simulink model "PV_SYSTEM_WITH_VARIOUS_MPPT"  (R2017a)
(part 5 of 6)

Energy-Tech (Zhejiang) ZSB-M270(156) | Solarbest Energy-Tech (Zhejiang) ZSB-P270(156) | Solarbest Energy-Tech (Zhejiang) SE-M275(156) | Solarbest Energy-Tech (Zhejiang) SE-P275(156) | Solarbest Energy-Tech (Zhejiang) ZSB-M275(156) | Solarbest Energy-Tech (Zhejiang) ZSB-P275(156) | Solarbest Energy-Tech (Zhejiang) SE-M280(156) | Solarbest Energy-Tech (Zhejiang) SE-P280(156) | Solarbest Energy-Tech (Zhejiang) ZSB-M280(156) | Solarbest Energy-Tech (Zhejiang) ZSB-P280(156) | Solarbest Energy-Tech (Zhejiang) SE-M285(156) | Solarbest Energy-Tech (Zhejiang) SE-P285(156) | Solarbest Energy-Tech (Zhejiang) ZSB-M285(156) | Solarbest Energy-Tech (Zhejiang) ZSB-P285(156) | Solarbest Energy-Tech (Zhejiang) SE-M290(156) | Solarbest Energy-Tech (Zhejiang) SE-P290(156) | Solarbest Energy-Tech (Zhejiang) ZSB-M290(156) | Solarbest Energy-Tech (Zhejiang) ZSB-P290(156) | Solarbest Energy-Tech (Zhejiang) SE-M295(156) | Solarbest Energy-Tech (Zhejiang) SE-P295(156) | Solarbest Energy-Tech (Zhejiang) ZSB-M295(156) | Solarbest Energy-Tech (Zhejiang) ZSB-P295(156) | Solarbest Energy-Tech (Zhejiang) SE-M300(156) | Solarbest Energy-Tech (Zhejiang) SE-P300(156) | Solarbest Energy-Tech (Zhejiang) ZSB-M300(156) | Solarbest Energy-Tech (Zhejiang) ZSB-P300(156) | Solarbest Energy-Tech (Zhejiang) SE-M305(156) | Solarbest Energy-Tech (Zhejiang) SE-P305(156) | Solarbest Energy-Tech (Zhejiang) ZSB-M305(156) | Solarbest Energy-Tech (Zhejiang) ZSB-P305(156) | Solarbest Energy-Tech (Zhejiang) SE-P310(156) | Solarbest Energy-Tech (Zhejiang) ZSB-P310(156) | Solarbine SB-S240TA1 | Solarbine SB-S245TA1 | Solarbine SB-S250TA1 | Solarbine S6T AC | Solarbine SB-S255TA1 | Solarbine SB-S260TA1 | Solarbine SB-S360TA1 | Solarbine SB-M365NA1 | Solarbine SB-S365TA1 | Solarbine SB-M370NA1 | Solarbine SB-S370TA1 | Solarbine SB-M375NA1 | Solarbine SB-S375TA1 | Solarbine SB-M380NA1 | Solarbine SB-S380SA1 | Solarbine SB-S380TA1 | Solarbine SB-M385NA1 | Solarbine SB-S385SA1 | Solarbine SB-S385TA1 | Solarbine SB-M390NA1 | Solarbine SB-S390SA1 | Solarbine SB-S390TA1 | Solarbine SB-M395NA1 | Solarbine SB-S395SA1 | Solarbine SB-S400SA1 | Solarbine SB-S405SA1 | Solarbine SB-S410SA1 | Solarbine SB-S415SA1 | Solarbine SB-S420SA1 | Solarfennel PS6A-230 | Solarfennel PS6A-235 | Solarfennel PS6A-240 | Solarfennel PS6A-245 | Solarfennel MS9A-250 | Solarfennel PS6A-250 | Solarfennel MS9A-255 | Solarfennel MS9A-260 | Solarfennel MS9A-265 | Solarfennel PS7A-270 | Solarfennel PS7A-275 | Solarfennel PS7A-280 | Solarfennel PS7A-285 | Solarfennel PS7A-290 | Solarfun Power SF220-30-P230 | Solarfun Power SF220-30-P235 | Solarfun Power SF220-30-P240 | Solargate Technology SG-2150 | Solargate Technology SG-2200 | Solargate Technology SG-2250 | Solargate Technology SG-2300 | Solargate Technology SG-2350 | Solaria Solaria 210 | Solaria Solaria 210 Frameless | Solaria Solaria 220 | Solaria Solaria 220 Frameless | Solaria Solaria 225 | Solaria Solaria 225 Frameless | Solaria Solaria 230 | Solaria Solaria 230 Frameless | Solaria Solaria 240 | Solaria Solaria 245 | Solaria Solaria 250 | Solaria Solaria 255 | Solaria Solaria 260 | Solaria Solaria 265 | Solaria Solaria 270 | Solaria Solaria 275 | Solaria Solaria 280 | Solarland USA SLP115S-17H | Solarland USA SLP120S-17H | Solarland USA SLP125S-17H | Solarland USA SLP160S-24H | Solarland USA SLP165S-24H | Solarland USA SLP170S-24H | Solarland USA SLP175S-24H | Solarland USA SLP175S-24J | Solarland USA SLP180S-24H | Solarland USA SLP180S-24J | Solarland USA SLP185S-24H | Solarland USA SLP185S-24J | Solarland USA SLP185S-72 | Solarland USA SLP190S-24H | Solarland USA SLP190S-72 | Solarland USA SLP195S-24H | Solarland USA SLP200-18H | Solarland USA SLP200S-24H | Solarland USA SLP205-18H | Solarland USA SLP210-18H | Solarland USA SLP215-18H | Solarland USA SLP215-60 | Solarland USA SLP220-18H | Solarland USA SLP220-60 | Solarland USA SLP225-60 | Solarland USA SLP230-18H | Solarland USA SLP230-60 | Solarland USA SLP230S-96 | Solarland USA SLP235-18H | Solarland USA SLP235-60 | Solarland USA SLP240-18H | Solarland USA SLP240S-96 | Solarland USA SLP245S-96 | Solarland USA SLP250S-96 | SolarPark Korea SPP 220 | SolarPark Korea SPP 225 | SolarPark Korea SPP 230 | SolarPark Korea SPP235 | SolarPark Korea SPP240 | SolarPark Korea SPP245 | SolarPark Korea SPP245 mono | SolarPark Korea SPP 250 | SolarPark Korea SPP250 mono | SolarPark Korea SPP255 mono | SolarPark Korea SPP260 mono | Solarpeace P6Y-230 | Solarpeace P6Y-235 | Solarpeace P6Y-240 | Solarpeace P6Y-245 | Solarpeace M9X-250 | Solarpeace P6Y-250 | Solarpeace M9X-255 | Solarpeace M9X-260 | Solarpeace M9X-265 | Solarpeace P7Y-270 | Solarpeace P7Y-275 | Solarpeace P7Y-280 | Solarpeace P7Y-285 | Solarpeace P7Y-290 | Solartec USA SDM-170-(165)-72M | Solartec USA SDM-170-(170)-72M | Solartec USA SDM-170-(175)-72M | Solartec USA SDM-170-(180)-72M | Solartec USA SDM-170-(185)-72M | Solartec S72MC-195 | Solartec S60MC-250 | Solartec S72PC-280 | Solartec S72MC6-300 | Solartech Energy ASC-6P-36-130 | Solartech Energy ASC-6P-36-135 | Solartech Energy ASC-6P-36-140 | Solartech Energy ASC-6P-36-145 | Solartech Energy ASC-6P-36-150 | Solartech Energy ASC-6P-48-175 | Solartech Energy ASC-6P-48-180 | Solartech Energy ASC-6P-48-185 | Solartech Energy ASC-6P-48-190 | Solartech Energy ASC-6P-48-195 | Solartech Energy ASC-6P-48-200 | Solartech Energy ASC-6P-54-200 | Solartech Energy ASC-6P-54-205 | Solartech Energy ASC-6P-54-210 | Solartech Energy SEC-210W-M6-G | Solartech Energy ASC-6P-54-215 | Solartech Energy SEC-215W-M6-G | Solartech Energy ASC-6P-54-220 | Solartech Energy ASC-6P-60-220 | Solartech Energy SEC-220W-M6-G | Solartech Energy SEC-6P-60-220 | Solartech Energy ASC-6P-54-225 | Solartech Energy ASC-6P-60-225 | Solartech Energy SEC-225W-M6-G | Solartech Energy SEC-6P-60-225 | Solartech Energy ASC-6P-54-230 | Solartech Energy ASC-6P-60-230 | Solartech Energy SEC-230W-M6-G | Solartech Energy SEC-6P-60-230 | Solartech Energy ASC-6P-60-235 | Solartech Energy SEC-6P-60-235 | Solartech Energy ASC-6P-60-240 | Solartech Energy SEC-6P-60-240 | Solartech Energy ASC-6P-60-245 | Solartech Energy SEC-6P-60-245 | Solartech Energy ASC-6P-60-250 | Solartech Energy ASC-6P-60-255 | Solartech Energy ASC-6P-72-265 | Solartech Energy ASC-6P-72-270 | Solartech Energy ASC-6P-72-275 | Solartech Energy ASC-6P-72-280 | Solartech Energy ASC-6P-72-285 | Solartech Energy ASC-6P-72-290 | Solartech Energy ASC-6P-72-295 | Solartech Energy ASC-6P-72-300 | Solartech Energy ASC-6P-72-305 | Solartech Power SPM190P | Solartech Power SPM195P | Solartech Power SPM200P | Solartech Power SPM205P | Solartech Power SPM210P | Solartech Power SPM220P | Solartech Power SPM225P | Solartech Power SPM230P | Solartech Power SPM235P | Solartech Power SPM240P | Solartech Renewables STR205 | Solartech Renewables STR210 | Solartech Renewables STR215 | Solartech Renewables STR220 | Solartech Renewables STR225 | Solartech Renewables STR230 | Solartechnics North America MP165Wp | Solartechnics North America Mp170Wp | Solartechnics North America MP175Wp | Solartechnics North America MP180Wp | SolarWorld SW165 mono | SolarWorld SW175 mono | SolarWorld SW220 mono | SolarWorld SW220 mono black | SolarWorld SW220 Poly | SolarWorld SW225 mono | SolarWorld SW225 mono black | SolarWorld SW225 Poly | SolarWorld SW230 mono | SolarWorld SW230 mono black | SolarWorld SW230 Poly | SolarWorld SW235 mono | SolarWorld SW235 mono black | SolarWorld SW235 Poly | SolarWorld SW240 mono | SolarWorld SW240 mono black | SolarWorld SW240 Poly | SolarWorld SW245 mono | SolarWorld SW245 Mono Black | SolarWorld SW245 Poly | SolarWorld SW250 Mono | SolarWorld SW250 Mono Black | SolarWorld SW250 Poly | SolarWorld Protect SW 255 Mono | SolarWorld Protect SW 255 Mono Black | SolarWorld SW255 Mono | SolarWorld SW255 Mono Black | SolarWorld SW255 Poly | SolarWorld Protect SW 260 Mono | SolarWorld Protect SW 260 Mono Black | SolarWorld SW260 Mono | SolarWorld SW260 Mono Black | SolarWorld Protect SW 265 Mono | SolarWorld Protect SW 265 Mono Black | SolarWorld SW265 Mono | SolarWorld SW265 Mono Black | SolarWorld Protect SW 270 Mono | SolarWorld Protect SW 270 Mono Black | SolarWorld SW270 Mono | SolarWorld SW270 Mono Black | SolarWorld Protect SW 275 Mono | SolarWorld SW275 Mono | Solarzentrum Allgau Wiosun A-170P | Solarzentrum Allgau Wiosun PVT 170 | Solarzentrum Allgau Wiosun A-175P | Solarzentrum Allgau Wiosun PVT 175 | Solarzentrum Allgau Wiosun A-180P | Solarzentrum Allgau Wiosun PVT 180 | Solarzentrum Allgau Wiosun A-185P | Solarzentrum Allgau Wiosun PVT 185 | Solarzentrum Allgau Wiosun A-190P | Solarzentrum Allgau Wiosun PVT 190 | SOLON SOLON Blue 220-01 215 | SOLON SOLON Blue 220 | SOLON SOLON Blue 220-01 220 | SOLON SOLON Black 225 | SOLON SOLON Black 230-01 225 | SOLON SOLON Black 230-15 225 | SOLON SOLON Blue 220-01 225 | SOLON SOLON Blue 225 | SOLON SOLON Corvus 225 | SOLON SOLON Black 230 | SOLON SOLON Black 230-01 230 | SOLON SOLON Black 230-15 230 | SOLON SOLON Blue 220-01 230 | SOLON SOLON Blue 230 | SOLON SOLON Corvus 230 | SOLON SOLON Black 230-01 235 | SOLON SOLON Black 230-15 235 | SOLON SOLON Black 235 | SOLON SOLON Blue 220-01 235 | SOLON SOLON Blue 235 | SOLON SOLON Corvus 235 | SOLON SOLON Black 230-01 240 | SOLON SOLON Black 230-15 240 | SOLON SOLON Black 240 | SOLON SOLON Blue 220-01 240 | SOLON SOLON Blue 240 | SOLON SOLON Corvus 240 | SOLON SOLON Black 245 | SOLON SOLON Blue 270-09 250 | SOLON SOLON Blue 270-09 255 | SOLON SOLON Blue 270-09 260 | SOLON SOLON Black 280-09 265 | SOLON SOLON Blue 270-09 265 | SOLON SOLON Blue XT 265 | SOLON SOLON Black 280-09 270 | SOLON SOLON Blue 270-09 270 | SOLON SOLON Blue XT 270 | SOLON SOLON Black 280-09 275 | SOLON SOLON Black XT 275 | SOLON SOLON Blue 270-09 275 | SOLON SOLON Blue XT 275 | SOLON SOLON Black 280-09 280 | SOLON SOLON Black XT 280 | SOLON SOLON Blue 270-09 280 | SOLON SOLON Blue XT 280 | SOLON SOLquick Black XT 280 | SOLON SOLquick Blue XT 280 | SOLON SOLquick Blue XT-H 280 | SOLON SOLON Black 280-09 285 | SOLON SOLON Black XT 285 | SOLON SOLON Blue 270-09 285 | SOLON SOLON Blue XT 285 | SOLON SOLquick Black XT 285 | SOLON SOLquick Blue XT 285 | SOLON SOLON Black 280-09 290 | SOLON SOLON Black XT 290 | SOLON SOLON Blue 270-09 290 | SOLON SOLquick Black XT 290 | SOLON SOLON Black 280-09 295 | SOLON SOLON Black XT 295 | SOLON SOLquick Black XT 295 | SOLON SOLON Black 280-09 300 | Solon SOLquick Black XT 300 | Solvation Manufacturing P6Y-230 | Solvation Manufacturing P6Y-235 | Solvation Manufacturing P6Y-240 | Solvation Manufacturing SM240-5M | Solvation Manufacturing SM240M-B | Solvation Manufacturing P6Y-245 | Solvation Manufacturing SM245-5M | Solvation Manufacturing SM245M-B | Solvation Manufacturing SM245M-Bv | Solvation Manufacturing SM245S-B | Solvation Manufacturing M9X-250 | Solvation Manufacturing P6Y-250 | Solvation Manufacturing SM250-5M | Solvation Manufacturing SM250M-B | Solvation Manufacturing SM250M-Bv | Solvation Manufacturing SM250S-B | Solvation Manufacturing M9X-255 | Solvation Manufacturing SM255-5M | Solvation Manufacturing SM255M-B | Solvation Manufacturing SM255M-Bv | Solvation Manufacturing SM255S-B | Solvation Manufacturing M9X-260 | Solvation Manufacturing SM260-5M | Solvation Manufacturing SM260M-Bv | Solvation Manufacturing M9X-265 | Solvation Manufacturing SM265M-Bv | Solvation Manufacturing P7Y-270 | Solvation Manufacturing SM270M-A | Solvation Manufacturing P7Y-275 | Solvation Manufacturing SM275M-A | Solvation Manufacturing P7Y-280 | Solvation Manufacturing SM280M-A | Solvation Manufacturing P7Y-285 | Solvation Manufacturing SM285M-A | Solvation Manufacturing SM285M-Av | Solvation Manufacturing P7Y-290 | Solvation Manufacturing SM290M-A | Solvation Manufacturing SM290M-Av | Solvation Manufacturing SM295M-A | Solvation Manufacturing SM295M-Av | Solvation Manufacturing SM300M-A | Solvation Manufacturing SM300M-Av | Solvation Manufacturing SM305M-A | Solvation Manufacturing SM305M-Av | Solvation Manufacturing SM310M-Av | Solvation Manufacturing SM315M-Av | Sonali Energees USA SS 1200 P | Sonali Energees USA SS 1250 P | Sonali Energees USA SS 1300 P | Sonali Energees USA SS 1400 P | Sonali Energees USA SS1750-170W | Sonali Energees USA SS 1750 P | Sonali Energees USA SS1750-175W | Sonali Energees USA SS 1800 P | Sonali Energees USA SS1750-180W | Sonali Energees USA SS 1900 P | Sonali Energees USA SS 2000 P | Sonali Energees USA SS 2100 P | Sonali Energees USA SS2100-210W | Sonali Energees USA SS2100-215W | Sonali Energees USA SS 2200 P | Sonali Energees USA SS2100-220W | Sonali Energees USA SS 2300 P | Sonali Energees USA SS2300-230W | Sonali Energees USA SS2300-235W | Sonali Energees USA SS 2400 P | Sonali Energees USA SS2300-240W | Sonali Energees USA SS2500-250W | Sonali Energees USA SS2800-275W | Sonali Energees USA SS2800-280W | Sonali Energees USA SS2800-285W | Sonali Energees SS 270 | Sonali Energees SS 280 | Sonali Energees SS 290 | Sonnetek SNK-165PSD | Sonnetek SNK-170PSD | Sonnetek SNK-175PSD | Sonnetek SNK-180PSD | Sonnetek SNK-250PSP | Sonnetek SNK-260PSP | Sonnetek SNK-270PSP | Sopray Energy SR-150 | Sopray Energy SR-160 | Sopray Energy SR-165 | Sopray Energy SR-170 | Sopray Energy SR-175 | Sopray Energy SR-180 | Sopray Energy SR156P-200 | Sopray Energy SR156P-210 | Sopray Energy SR156P-220 | Sopray Energy SR156P-230 | Sova Power SOLARSOVA 200P | Sova Power SOLARSOVA 205P | Sova Power SOLARSOVA 210P | Sova Power SOLARSOVA 215P | Sova Power SOLARSOVA 220P | Sova Power SOLARSOVA 235P | Sova Power SOLARSOVA 240P | Sova Power SOLARSOVA 245P | Sova Power SOLARSOVA 250P | Sova Power SOLARSOVA 255P | Sova Power SOLARSOVA 260P | Sovello SV-T-190-yyy | Sovello SV-X-190-yyy | Sovello SV-T-195-yyy | Sovello SV-X-195-yyy | Sovello SV-T-200-yyy | Sovello SV-X-200-yyy | Sovello SV-X-205-yyy | Sovello SV-X-210-yyy | SRS Energy SPT16 | Star Harvest Solar SHS260-5M | Stion SN-110 | Stion STN-110 | Stion SN-115 | Stion STN-115 | Stion SN-120 | Stion STN-120 | Stion SN-125 | Stion STN-125 | Stion STX-125 | Stion SN-130 | Stion STN-130 | Stion STX-130 | Stion SN-135 | Stion STN-135 | Stion STX-135 | Stion SN-140 | Stion STN-140 | Stion STX-140 | Stion SN-145 | Stion STN-145 | Stion STX-145 | Stion SN-150 | Stion STN-150 | STX Solar STX-240MT2 | STX Solar STX-245MT2 | STX Solar STX-250MT2 | STX Solar STX-255MT2 | STX Solar STX-260MT2 | STX Solar STX-290MT2 | STX Solar STX-295MT2 | STX Solar STX-300MT2 | STX Solar STX-305MT2 | Sun Earth Solar Power TDB125x125-36-P 80W | Sun Earth Solar Power TDB125x125-36-P 85W | Sun Earth Solar Power TPB125x125-36-P 85W | Sun Earth Solar Power TDB125x125-36-P 90W | Sun Earth Solar Power TPB125x125-36-P 90W | Sun Earth Solar Power TDB125x125-36-P 95W | Sun Earth Solar Power TPB125x125-36-P 95W | Sun Earth Solar Power TDB156x156-36-P 125W | Sun Earth Solar Power TPB156x156-36-P 125W | Sun Earth Solar Power TDB156x156-36-P 130W | Sun Earth Solar Power TPB156x156-36-P 130W | Sun Earth Solar Power TDB156x156-36-P 135W | Sun Earth Solar Power TPB156x156-36-P 135W | Sun Earth Solar Power TDB156x156-36-P 140W | Sun Earth Solar Power TPB156x156-36-P 140W | Sun Earth Solar Power TDB156x156-36-P 145W | Sun Earth Solar Power TPB156x156-36-P 145W | Sun Earth Solar Power TDB125x125-72-P 150W | Sun Earth Solar Power TPB125x125-72-P 150W | Sun Earth Solar Power TDB125x125-72-P 155W | Sun Earth Solar Power TPB125x125-72-P 155W | Sun Earth Solar Power TDB125x125-72-P 160W | Sun Earth Solar Power TPB125x125-72-P 160W | Sun Earth Solar Power TDB125x125-72-P 165W | Sun Earth Solar Power TPB125x125-72-P 165W | Sun Earth Solar Power TDB125x125-72-P 170W | Sun Earth Solar Power TPB125x125-72-P 170W | Sun Earth Solar Power TDB125x125-72-P 175W | Sun Earth Solar Power TPB125x125-72-P 175W | Sun Earth Solar Power TDB125x125-72-P 180W | Sun Earth Solar Power TPB125x125-72-P 180W | Sun Earth Solar Power TPB156x156-54-P 180W | Sun Earth Solar Power TDB125x125-72-P 185W | Sun Earth Solar Power TPB125x125-72-P 185W | Sun Earth Solar Power TPB156x156-54-P 185W | Sun Earth Solar Power TDB125x125-72-P 190W | Sun Earth Solar Power TPB125x125-72-P 190W | Sun Earth Solar Power TPB156x156-54-P 190W | Sun Earth Solar Power TPB156x156-54-P 195W | Sun Earth Solar Power TPB125x125-96-P 200W | Sun Earth Solar Power TPB156x156-54-P 200W | Sun Earth Solar Power TPB156x156-60-P 200W | Sun Earth Solar Power TPB156x156-54-P 205W | Sun Earth Solar Power TPB156x156-60-P 205W | Sun Earth Solar Power TPB125x125-96-P 210W | Sun Earth Solar Power TPB156x156-54-P 210W | Sun Earth Solar Power TPB156x156-60-P 210W | Sun Earth Solar Power TDB156x156-60-P 215W | Sun Earth Solar Power TPB156x156-54-P 215W | Sun Earth Solar Power TPB156x156-60-P 215W | Sun Earth Solar Power TDB156x156-60-P 220W | Sun Earth Solar Power TPB125x125-96-P 220W | Sun Earth Solar Power TPB156x156-54-P 220W | Sun Earth Solar Power TPB156x156-60-P 220W | Sun Earth Solar Power TDB156x156-60-P 225W | Sun Earth Solar Power TPB156x156-60-P 225W | Sun Earth Solar Power TDB156x156-60-P 230W | Sun Earth Solar Power TPB125x125-96-P 230W | Sun Earth Solar Power TPB156x156-60-P 230W | Sun Earth Solar Power TPB156x156-72-P 230W | Sun Earth Solar Power TDB156x156-60-P 235W | Sun Earth Solar Power TPB156x156-60-P 235W | Sun Earth Solar Power TDB156x156-60-P 240W | Sun Earth Solar Power TPB125x125-96-P 240W | Sun Earth Solar Power TPB156x156-60-P 240W | Sun Earth Solar Power TPB156x156-72-P 240W | Sun Earth Solar Power TDB156x156-60-P 245W | Sun Earth Solar Power TPB156x156-60-P 245W | Sun Earth Solar Power TPB156x156-72-P 250W | Sun Earth Solar Power TPB156x156-72-P 255W | Sun Earth Solar Power TPB156x156-72-P 260W | Sun Earth Solar Power TPB156x156-72-P 270W | Sun Earth Solar Power TDB156x156-72-P 280W | Sun Earth Solar Power TPB156x156-72-P 280W | Sun Earth Solar Power TDB156x156-72-P 285W | Sun Earth Solar Power TPB156x156-72-P 285W | Sun Earth Solar Power TDB156x156-72-P 290W | Sun Earth Solar Power TPB156x156-72-P 290W | Sun Earth Solar Power TDB156x156-72-P 295W | Sun Earth Solar Power TPB156x156-72-P 295W | Sun Energy Engineering SE14-50 | Sun Energy Engineering SE14-52 | Sun World Solar Energy Technology (Luoyang) SWM230P156 | Sun World Solar Energy Technology (Luoyang) SWM235M156 | Sun World Solar Energy Technology (Luoyang) SWM235P156 | Sun World Solar Energy Technology (Luoyang) SWM240M156 | Sun World Solar Energy Technology (Luoyang) SWM240P156 | Sun World Solar Energy Technology (Luoyang) SWM245M156 | Sun World Solar Energy Technology (Luoyang) SWM245P156 | Sun World Solar Energy Technology (Luoyang) SWM250M156 | Sun World Solar Energy Technology (Luoyang) SWM250P156 | Sun World Solar Energy Technology (Luoyang) SWM255M156 | Sun World Solar Energy Technology (Luoyang) SWM280P156 | Sun World Solar Energy Technology (Luoyang) SWM285M156 | Sun World Solar Energy Technology (Luoyang) SWM285P156 | Sun World Solar Energy Technology (Luoyang) SWM290M156 | Sun World Solar Energy Technology (Luoyang) SWM290P156 | Sun World Solar Energy Technology (Luoyang) SWM295M156 | Sun World Solar Energy Technology (Luoyang) SWM295P156 | Sun World Solar Energy Technology (Luoyang) SWM300M156 | Sun World Solar Energy Technology (Luoyang) SWM300P156 | Sunarray SUNARRAY-M6B2409-130 | Sunarray SUNARRAY-M6B2409-135 | Sunarray SUNARRAY-S6B2409-135 | Sunarray SUNARRAY-M6B2409-140 | Sunarray SUNARRAY-S6B2409-140 | Sunarray SUNARRAY-S6B2409-145 | Sunarray SUNARRAY-M6B2608-175 | Sunarray SUNARRAY-M6B2608-180 | Sunarray SUNARRAY-S6B2608-180 | Sunarray SUNARRAY-M6B2608-185 | Sunarray SUNARRAY-S6B2608-185 | Sunarray SUNARRAY-M6B2609-190 | Sunarray SUNARRAY-S6B2608-190 | Sunarray SUNARRAY-M6B2609-195 | Sunarray SUNARRAY-S6B2609-195 | Sunarray SUNARRAY-M6B2609-200 | Sunarray SUNARRAY-S6B2609-200 | Sunarray SUNARRAY-M6B2609-205 | Sunarray SUNARRAY-S6B2609-205 | Sunarray SUNARRAY-M6B2609-210 | Sunarray SUNARRAY-S6B2609-210 | Sunarray SUNARRAY-M6B2609-215 | Sunarray SUNARRAY-S6B2609-215 | Sunarray SUNARRAY-M6B2609-220 | Sunarray SUNARRAY-S6B2609-220 | Sunarray SUNARRAY-M6B2609-225 | Sunarray SUNARRAY-S6B2609-225 | Sunarray SUNARRAY-M6B2609-230 | Sunarray SUNARRAY-S6B2609-230 | Sunarray SUNARRAY-M6B2610-235 | Sunarray SUNARRAY-S6B2609-235 | Sunarray SUNARRAY-M6B2610-240 | Sunarray SUNARRAY-S6B2609-240 | Sunarray SUNARRAY-M6B3612-270T | Sunarray SUNARRAY-M6B2612-275 | Sunarray SUNARRAY-M6B3612-275T | Sunarray SUNARRAY-M6B2612-280 | Sunarray SUNARRAY-M6B3612-280T | Sunarray SUNARRAY-M6B2612-285 | Sunarray SUNARRAY-M6B3612-285T | Sunarray SUNARRAY-S6B3612-285T | Sunarray SUNARRAY-M6B2612-290 | Sunarray SUNARRAY-M6B3612-290T | Sunarray SUNARRAY-S6B3612-290T | Sunarray SUNARRAY-M6B2612-295 | Sunarray SUNARRAY-S6B3612-295T | Sunarray SUNARRAY-S6B3612-300T | Sunarray SUNARRAY-S6B3612-305T | SUNGEN International SG-HN90-GG | SUNGEN International SG-HN95-GG | SUNGEN International SG-HN100-GG | SUNGEN International SG-HN105-GG | SUNGEN International SG-HN110-GG | SUNGEN International SGM-160D | SUNGEN International SGM-165D | SUNGEN International SGM-170D | SUNGEN International SGM-175D | SUNGEN International SGM-180D | SUNGEN International SGM-185D | SUNGEN International SGM-190D | SUNGEN International SGM-195D | SUNGEN International SGM-200D | SUNGEN International SGM-200P | SUNGEN International SGM-205D | SUNGEN International SGM-205P | SUNGEN International SGM-210D | SUNGEN International SGM-210P | SUNGEN International SGM-215D | SUNGEN International SGM-215P | SUNGEN International SGM-220D | SUNGEN International SGM-220P | SUNGEN International SGM-225D | SUNGEN International SGM-225P | SUNGEN International SGM-230D | SUNGEN International SGM-230P | SUNGEN International SGM-235D | SUNGEN International SGM-235P | SUNGEN International SGM-240D | SUNGEN International SGM-240P | SUNGEN International SGM-245D | SUNGEN International SGM-245P | SUNGEN International SGM-250D | SUNGEN International SGM-250P | SUNGEN International SGM-255P | SUNGEN International SGM-260D | SUNGEN International SGM-260P | SUNGEN International SGM-265P | SUNGEN International SGM-270P | SUNGEN International SGM-275P | SUNGEN International SGM-280P | SUNGEN International SGM-285P | Suniva MVS220-60-5-501 | Suniva MVS225-60-5-501 | Suniva ART230-60-3-100 | Suniva MVP230-60-5-401 | Suniva MVS230-60-5-501 | Suniva ART235-60-3-100 | Suniva ART235-60-3-101 | Suniva ART235-60-3-1B0 | Suniva MVP235-60-5-401 | Suniva MVS235-60-5-501 | Suniva MVT235-60-5-100 | Suniva MVX235-60-5-701 | Suniva OPT235-60-4-100 | Suniva OPT235-60-4-1B0 | Suniva ART240-60-3-100 | Suniva ART240-60-3-101 | Suniva ART240-60-3-1B0 | Suniva MVP240-60-5-401 | Suniva MVS240-60-5-501 | Suniva MVT240-60-5-100 | Suniva MVX240-60-5-701 | Suniva MVX240-60-5-7B1 | Suniva MVX240-60-5-801 | Suniva MVX240-60-5-8B1 | Suniva OPT240-60-4-100 | Suniva OPT240-60-4-1B0 | Suniva ART245-60-3-100 | Suniva ART245-60-3-101 | Suniva ART245-60-3-1B0 | Suniva MVT245-60-5-100 | Suniva MVX245-60-5-701 | Suniva MVX245-60-5-7B1 | Suniva MVX245-60-5-801 | Suniva MVX245-60-5-8B1 | Suniva OPT245-60-4-100 | Suniva OPT245-60-4-1B0 | Suniva ART250-60-3-100 | Suniva ART250-60-3-101 | Suniva ART250-60-3-1B0 | Suniva MVT250-60-5-100 | Suniva MVX250-60-5-701 | Suniva MVX250-60-5-7B1 | Suniva MVX250-60-5-801 | Suniva MVX250-60-5-8B1 | Suniva OPT250-60-4-100 | Suniva OPT250-60-4-1B0 | Suniva OPT250-60-4-700 | Suniva OPT250-60-4-7B0 | Suniva OPT250-60-4-800 | Suniva OPT250-60-4-8B0 | Suniva ART255-60-3-100 | Suniva ART255-60-3-1B0 | Suniva MVX255-60-5-701 | Suniva MVX255-60-5-7B1 | Suniva MVX255-60-5-801 | Suniva MVX255-60-5-8B1 | Suniva OPT255-60-4-100 | Suniva OPT255-60-4-1B0 | Suniva OPT255-60-4-700 | Suniva OPT255-60-4-7B0 | Suniva OPT255-60-4-800 | Suniva OPT255-60-4-8B0 | Suniva MVX260-60-5-7B1 | Suniva MVX260-60-5-801 | Suniva MVX260-60-5-8B1 | Suniva OPT260-60-4-100 | Suniva OPT260-60-4-1B0 | Suniva OPT260-60-4-700 | Suniva OPT260-60-4-7B0 | Suniva OPT265-60-4-100 | Suniva OPT265-60-4-1B0 | Suniva OPT270-60-4-100 | Suniva MVP280-72-5-401 | Suniva MVT280-72-5-100 | Suniva MVP285-72-5-401 | Suniva MVT285-72-5-100 | Suniva MVX285-72-5-701 | Suniva MVX285-72-5-801 | Suniva MVT290-72-5-100 | Suniva MVX290-72-5-701 | Suniva MVX290-72-5-801 | Suniva OPT290-72-4-100 | Suniva MVT295-72-5-100 | Suniva MVX295-72-5-701 | Suniva MVX295-72-5-801 | Suniva OPT295-72-4-100 | Suniva MVT300-72-5-100 | Suniva MVX300-72-5-701 | Suniva MVX300-72-5-801 | Suniva OPT300-72-4-100 | Suniva MVX305-72-5-701 | Suniva MVX305-72-5-801 | Suniva OPT305-72-4-100 | Suniva OPT305-72-4-800 | Suniva MVX310-72-5-801 | Suniva OPT310-72-4-100 | Suniva OPT310-72-4-800 | Suniva OPT315-72-4-100 | Suniva OPT315-72-4-800 | Suniva OPT320-72-4-800 | Sunlan Solar SLM225P | Sunlan Solar SLM230P | Sunlan Solar SLM235P | Sunlan Solar SLM240P | Sunlan Solar SLM245P | Sunlan Solar SLM270P | Sunlan Solar SLM275P | Sunlan Solar SLM280P | Sunny International Power SPM-180PB203 | Sunny International Power SPM-180SB105 | Sunny International Power SPM-190PB203 | Sunny International Power SPM-190SB105 | Sunny International Power SPM-200PB203 | Sunny International Power SPM-200PB204 | Sunny International Power SPM-200SB105 | Sunny International Power SPM-210PB203 | Sunny International Power SPM-210PB204 | Sunny International Power SPM-220PB203 | Sunny International Power SPM-220PB204 | Sunny International Power SPM-230PB204 | Sunny International Power SPM-230PB206 | Sunny International Power SPM-240PB204 | Sunny International Power SPM-240PB205 | Sunny International Power SPM-240PB206 | Sunny International Power SPM-250PB205 | Sunny International Power SPM-250PB206 | Sunny International Power SPM-260PB205 | Sunny International Power SPM-260PB206 | Sunny International Power SPM-270PB205 | Sunny International Power SPM-270PB206 | Sunny International Power SPM-280PB205 | Sunny International Power SPM-290PB205 | Sunny Optronics 7NACF00-06A225 | Sunny Optronics 7NACF00-06A230 | Sunny Optronics 7NACF00-06A235 | Sunny Optronics 7NACF00-06A240 | Sunny Optronics 7NACF00-06A245 | Sunperfect Solar CRM60S125M-24 | Sunperfect Solar CRM60S125S | Sunperfect Solar CRM85S125M-36 | Sunperfect Solar CRM85S125S | Sunperfect Solar CRM115S125M-48 | Sunperfect Solar CRM115S125S | Sunperfect Solar CRM145S125M-60 | Sunperfect Solar CRM145S125S | Sunperfect Solar CRM175S125M-72 | Sunperfect Solar CRM175S125S | Sunperfect Solar CRM180S125M-72 | Sunperfect Solar CRM185S125M-72 | Sunperfect Solar CRM185S156P-54 | Sunperfect Solar CRM190S125M-72 | Sunperfect Solar CRM190S156P-54 | Sunperfect Solar CRM195S125M-72 | Sunperfect Solar CRM195S125M-80 | Sunperfect Solar CRM195S125S | Sunperfect Solar CRM195S156P-54 | Sunperfect Solar CRM200S156P-54 | Sunperfect Solar CRM200S156P-60 | Sunperfect Solar CRM205S125M-80 | Sunperfect Solar CRM205S156P-54 | Sunperfect Solar CRM205S156P-60 | Sunperfect Solar CRM210S125M-80 | Sunperfect Solar CRM210S156P-54 | Sunperfect Solar CRM210S156P-60 | Sunperfect Solar CRM215S125M-80 | Sunperfect Solar CRM215S156P-54 | Sunperfect Solar CRM215S156P-60 | Sunperfect Solar CRM220S156P-54 | Sunperfect Solar CRM220S156P-60 | Sunperfect Solar CRM225S156P-54 | Sunperfect Solar CRM225S156P-60 | Sunperfect Solar CRM230S156P-54 | Sunperfect Solar CRM230S156P-60 | Sunperfect Solar CRM235S125M-96 | Sunperfect Solar CRM235S125S | Sunperfect Solar CRM235S156P-60 | Sunperfect Solar CRM240S125M-96 | Sunperfect Solar CRM240S156P-60 | Sunperfect Solar CRM240S156P-72 | Sunperfect Solar CRM245S125M-96 | Sunperfect Solar CRM245S156P-60 | Sunperfect Solar CRM245S156P-72 | Sunperfect Solar CRM250S125M-96 | Sunperfect Solar CRM250S156P-60 | Sunperfect Solar CRM250S156P-72 | Sunperfect Solar CRM255S125M-96 | Sunperfect Solar CRM255S156P-60 | Sunperfect Solar CRM255S156P-72 | Sunperfect Solar CRM260S125M-96 | Sunperfect Solar CRM260S156P-60 | Sunperfect Solar CRM260S156P-72 | Sunperfect Solar CRM265S125M-96 | Sunperfect Solar CRM265S156P-72 | Sunperfect Solar CRM270S156P-72 | Sunperfect Solar CRM275S156P-72 | Sunperfect Solar CRM280S156P-72 | Sunperfect Solar CRM285S156P-72 | Sunperfect Solar CRM290S156P-72 | Sunperfect Solar CRM295S156P-72 | Sunperfect Solar CRM300S156P-72 | SunPower PL-PLT-63L-BLK-U | SunPower SPR-76R-BLK-U | SunPower SPR-76RE-BLK-U | SunPower SPR-200-BLK-U | SunPower SPR-200-WHT-U | SunPower SPR-205-BLK-U | SunPower SPR-208-WHT-U | SunPower SPR-210-BLK-U | SunPower SPR-210-WHT-U | SunPower PL-SUNP-SPR-215 | SunPower SPR-215-WHT-U | SunPower SPR-217-WHT-U | SunPower SER-220P | SunPower SPR-220-BLK-U | SunPower SPR-220-WHT-U | SunPower SPR-225-BLK-U | SunPower SPR-225E-BLK-D | SunPower SPR-225E-BLK-U-ACPV | SunPower SPR-225E-WHT-D | SunPower SPR-225NE-BLK-D | SunPower SER-228P | SunPower SPR-230E-WHT-D | SunPower SPR-230NE-BLK-D | SunPower SPR-230NE-BLK-U-ACPV | SunPower SPR-230-WHT-U | SunPower SER-235P | SunPower SPR-235NE-WHT-D | SunPower SPR-E19-235 | SunPower T5-SER-235P | SunPower SPR-238E-WHT-D | SunPower SPR-240E-WHT-D | SunPower SPR-240E-WHT-U-ACPV | SunPower SPR-E19-240 | SunPower SPR-245NE-WHT-D | SunPower SPR-245NE-WHT-U-240 ACPV | SunPower SPR-245NE-WHT-U-ACPV | SunPower SPR-E19-245 | SunPower SPR-E20-245 | SunPower SPR-E20-245-A-AC | SunPower SPR-X20-245 | SunPower SPR-250NX-BLK-D | SunPower SPR-X20-250-BLK | SunPower SPR-X20-250-BLK-A-AC | SunPower SPR-X20-250-BLK-LAM | SunPower SPR-X20-255 | SunPower SPR-X21-255 | SunPower PL-SUNP-SPR-290 | SunPower SPR-290-WHT-U | SunPower T5-SPR-290 | SunPower SPR-295E-WHT-D | SunPower SPR-295E-WHT-U | SunPower SPR-E18-295-COM | SunPower SPR-300E-WHT-D | SunPower SPR-300NE-WHT-D | SunPower SPR-E18-300-COM | SunPower PL-SUNP-SPR-305 | SunPower SPR-305E-WHT-D | SunPower SPR-305E-WHT-U | SunPower SPR-305NE-WHT-D | SunPower SPR-305-WHT-U | SunPower SPR-E18-305-COM | SunPower T5-SPR-305 | SunPower T5-SPR-305E | SunPower PL-SUNP-SPR-308E | SunPower SPR-308E-WHT-D | SunPower SPR-308NE-WHT-D | SunPower T5-SPR-308E | SunPower PL-SUNP-SPR-310 | SunPower SPR-310E-WHT-D | SunPower SPR-310E-WHT-U | SunPower SPR-310-WHT-U | SunPower SPR-E19-310-COM | SunPower T5-SPR-310 | SunPower PL-SUNP-SPR-315E | SunPower SPR-315E-WHT-D | SunPower SPR-315E-WHT-U | SunPower SPR-315NE-WHT-D | SunPower SPR-E19-315 | SunPower SPR-E19-315-COM | SunPower T5-SPR-315 | SunPower T5-SPR-315E | SunPower PL-SUNP-SPR-318E | SunPower SPR-318E-WHT-D | SunPower T5-SPR-318E | SunPower SPR-320E-WHT-D | SunPower SPR-320NE-WHT-D | SunPower SPR-E19-320 | SunPower SPR-E19-320-COM | SunPower T5-SPR-320E | SunPower SPR-327NE-WHT-D | SunPower SPR-E20-327 | SunPower SPR-E20-327-COM | SunPower SPR-E20-327-COM-LAM | SunPower SPR-E20-327-COM-T5 | SunPower SPR-X20-327 | SunPower SPR-X20-327-BLK | SunPower SPR-X20-327-COM | SunPower T5-SPR-327 | SunPower SPR-335NX-BLK-D | SunPower SPR-X21-335 | SunPower SPR-X21-335-BLK | SunPower SPR-343J-WHT-D | SunPower SPR-343NJ-WHT-D | SunPower SPR-343NX-BLK-D | SunPower SPR-343NX-WHT-D | SunPower SPR-X21-345 | SunPower SPR-X21-345-COM | SunPower SPR-390E-WHT-D | SunPower SPR-400E-WHT-D | SunPower SPR-410NE-WHT-D | SunPower SPR-E19-410-COM | SunPower SPR-415E-WHT-D | SunPower SPR-425E-WHT-D | SunPower SPR-435NE-WHT-D | SunPower SPR-E20-435-COM | SunPower SPR-440NE-WHT-D | SunPower SPR-445J-WHT-D | SunPower SPR-445NJ-WHT-D | SunPower SPR-445NX-WHT-D | SunPower SPR-X20-445-COM | Sunpreme Inc. SNPM-GX-72-245 | Sunpreme Inc. SNPM-GX-72-250 | Sunpreme Inc. SNPM-GX-72-255 | Sunpreme SNPM-F60-02-180 | Sunpreme SNPM-G60-02-180 | Sunpreme SNPM-F60-02-185 | Sunpreme SNPM-G60-02-185 | Sunpreme SNPM-F60-02-190 | Sunpreme SNPM-G60-02-190 | Sunpreme SNPM-G60-02-195 | Sunpreme SNPM-G60-02-200 | Sunpreme SNPM-G60-02-205 | Sunpreme SNPM-G60-02-210 | Sunpreme SNPM-G60-02-215 | Sunpreme SNPM-G60-02-220 | Sunpreme SNPM-GX-220 | Sunpreme SNPM-GX-225 | Sunpreme SNPM-GX-230 | Sunpreme SNPM-GX-235 | Sunpreme SNPM-GX-240 | Sunpreme SNPM-GX-285 | Sunpreme SNPM-GX-290 | Sunpreme SNPM-GX-295 | Sunpreme SNPM-GX-300 | Sunpreme SNPM-GX-305 | Sunpreme SNPM-GX-310 | Sunpreme SNPM-GX-315 | Sunrise Solartech SR-M572185 | Sunrise Solartech SR-M648185 | Sunrise Solartech SR-M572190 | Sunrise Solartech SR-M648190 | Sunrise Solartech SR-M572195 | Sunrise Solartech SR-M648195 | Sunrise Solartech SR-M572200 | Sunrise Solartech SR-M648200 | Sunrise Solartech SR-M572205 | Sunrise Solartech SR-M648205 | Sunrise Solartech SR-M654210 | Sunrise Solartech SR-M654215 | Sunrise Solartech SR-M654220 | Sunrise Solartech SR-P660220 | Sunrise Solartech SR-M654225 | Sunrise Solartech SR-P660225 | Sunrise Solartech SR-M654230 | Sunrise Solartech SR-P660230 | Sunrise Solartech SR-M660235 | Sunrise Solartech SR-P660235 | Sunrise Solartech SR-M660240 | Sunrise Solartech SR-P660240 | Sunrise Solartech SR-M660245 | Sunrise Solartech SR-M660250 | Sunrise Solartech SR-M660255 | Sunrise Solartech SR-M660260 | Sunrise Solartech SR-P672275 | Sunrise Solartech SR-M672280 | Sunrise Solartech SR-P672280 | Sunrise Solartech SR-M672285 | Sunrise Solartech SR-P672285 | Sunrise Solartech SR-M672290 | Sunrise Solartech SR-P672290 | Sunrise Solartech SR-M672295 | Sunrise Solartech SR-P672295 | Sunrise Solartech SR-M672300 | Sunrise Solartech SR-M672305 | Sunrise Solartech SR-M672310 | Suntech Power STP050D-5-ZCB | Suntech Power STP050D-5-ZCF | Suntech Power STP050D-5-ZCG | Suntech Power STP120D-12-VEC | Suntech Power STP130D-12-VEC | Suntech Power STP135D-12-VEC | Suntech Power STP160S-24-Ab-1 Black | Suntech Power STP165S-24-Ab-1 Black | Suntech Power STP170S-24-Ab-1 | Suntech Power STP170S-24-Ab-1 Black | Suntech Power STP170S-24-Ad+ | Suntech Power STP170S-24-Adb+ | Suntech Power MSZ175B-F | Suntech Power MSZ175J-F | Suntech Power STP175S-24-Ab-1 | Suntech Power STP175S-24-Ab-1 Black | Suntech Power STP175S-24-Ad+ | Suntech Power STP175S-24-Adb+ | Suntech Power MSZ180B-F | Suntech Power MSZ180J-F | Suntech Power STP180S-24-Ab-1 | Suntech Power STP180S-24-Ab-1 Black | Suntech Power STP180S-24-Ad+ | Suntech Power STP180S-24-Adb+ | Suntech Power STP185S-24-Ab-1 | Suntech Power STP185S-24-Ad+ | Suntech Power STP185S-24-Adb | Suntech Power STP185S-24-Adb+ | Suntech Power PLUTO190-Ada | Suntech Power PLUTO190-Adb | Suntech Power PLUTO190-Ade | Suntech Power PLUTO190-Adf | Suntech Power STP190-18-UB-1 | Suntech Power STP190S-24-Ad | Suntech Power STP190S-24-Ad+ | Suntech Power STP190S-24-Adb | Suntech Power STP190S-24-Adb+ | Suntech Power PLUTO195-Ada | Suntech Power PLUTO195-Adb | Suntech Power PLUTO195-Ade | Suntech Power PLUTO195-Adf | Suntech Power STP195S-24-Ad | Suntech Power STP195S-24-Ad+ | Suntech Power STP195S-24-Adb | Suntech Power STP195S-24-Adb+ | Suntech Power PLUTO200-Ada | Suntech Power PLUTO200-Adb | Suntech Power PLUTO200-Ade | Suntech Power PLUTO200-Adf | Suntech Power STP200-18-UB-1 | Suntech Power STP200-18-Ud | Suntech Power PLUTO205-Ada | Suntech Power PLUTO205-Adb | Suntech Power PLUTO205-Ade | Suntech Power PLUTO205-Adf | Suntech Power STP205-18-Ud | Suntech Power PLUTO210-Ada | Suntech Power PLUTO210-Adb | Suntech Power PLUTO210-Ade | Suntech Power PLUTO210-Adf | Suntech Power PLUTO210-Udm | Suntech Power STP210-18-UB-1 | Suntech Power STP210-18-Ud | Suntech Power STP210-20-Wd | Suntech Power STP210-20-Wde | Suntech Power PLUTO215-Udm | Suntech Power STP215-18-Ud | Suntech Power STP215-20-Wd | Suntech Power STP215-20-Wde | Suntech Power PLUTO220-Udm | Suntech Power STP220-18-Ud | Suntech Power STP220-20-Wd | Suntech Power STP220-20-Wde | Suntech Power STP220-20-Wdl | Suntech Power PLUTO225-Udm | Suntech Power STP225-18-Ud | Suntech Power STP225-20-Wd | Suntech Power STP225-20-Wde | Suntech Power STP225-20-Wdl | Suntech Power PLUTO230-Udm | Suntech Power PLUTO230-Wdb | Suntech Power PLUTO230-Wde | Suntech Power PLUTO230-Wdm | Suntech Power STP230-20-Wd | Suntech Power STP230-20-Wde | Suntech Power STP230-20-Wdl | Suntech Power STP230S-20-Wd | Suntech Power STP230S-20-Wdb | Suntech Power STP230S-20-Wde | Suntech Power PLUTO235-Wdb | Suntech Power PLUTO235-Wde | Suntech Power PLUTO235-Wdm | Suntech Power STP235-20-Wd | Suntech Power STP235-20-Wde | Suntech Power STP235-20-Wdl | Suntech Power STP235S-20-Wd | Suntech Power STP235S-20-Wdb | Suntech Power STP235S-20-Wde | Suntech Power PLUTO240-Wdb | Suntech Power PLUTO240-Wde | Suntech Power PLUTO240-Wdm | Suntech Power STP240-20-Wd | Suntech Power STP240-20-Wdb | Suntech Power STP240-20-Wde | Suntech Power STP240-20-Wdl | Suntech Power STP240S-20-Wd | Suntech Power STP240S-20-Wdb | Suntech Power STP240S-20-Wde | Suntech Power PLUTO245-Wdb | Suntech Power PLUTO245-Wde | Suntech Power PLUTO245-Wdm | Suntech Power STP245-20-Wd | Suntech Power STP245-20-Wdb | Suntech Power STP245-20-Wde | Suntech Power STP245S-20-Wd | Suntech Power STP245S-20-Wdb | Suntech Power STP245S-20-Wde | Suntech Power PLUTO250-Wdb | Suntech Power PLUTO250-Wde | Suntech Power PLUTO250-Wdm | Suntech Power STP250-20-Wd | Suntech Power STP250-20-Wdb | Suntech Power STP250-20-Wde | Suntech Power STP250D-24-VEC | Suntech Power STP250S-20-Wd | Suntech Power STP250S-20-Wdb | Suntech Power STP250S-20-Wde | Suntech Power STP255-20-Wd | Suntech Power STP255-20-Wdb | Suntech Power STP255-20-Wde | Suntech Power STP255S-20-Wdb | Suntech Power STP255S-20-Wde | Suntech Power STP260-20-Wd | Suntech Power STP260-20-Wdb | Suntech Power STP260-20-Wde | Suntech Power STP260-24-Vb-1 | Suntech Power STP260-24-Vd | Suntech Power STP260-24-Ve | Suntech Power STP260D-24-VEC | Suntech Power STP260S-20-Wdb | Suntech Power STP260S-20-Wde | Suntech Power STP260-VRM-1 | Suntech Power STP265-20-Wd | Suntech Power STP265-20-Wde | Suntech Power STP270-24-Vb-1 | Suntech Power STP270-24-Vd | Suntech Power STP270-24-Vdx | Suntech Power STP270-24-Ve | Suntech Power STP270D-24-VEC | Suntech Power STP270-VRM-1 | Suntech Power STP275-24-Vd | Suntech Power STP275-24-Vdx | Suntech Power STP275-24-Ve | Suntech Power STP275-VRM-1 | Suntech Power STP275-VRM-1.5 | Suntech Power PLUTO280-Vdm | Suntech Power PLUTO280-Vdx | Suntech Power STP280-24-Vb-1 | Suntech Power STP280-24-Vd | Suntech Power STP280-24-Vdx | Suntech Power STP280-24-Ve | Suntech Power STP280-VRM-1 | Suntech Power STP280-VRM-1.5 | Suntech Power PLUTO285-Vdm | Suntech Power PLUTO285-Vdx | Suntech Power STP285-24-Vd | Suntech Power STP285-24-Vdx | Suntech Power STP285-24-Ve | Suntech Power STP285-VRM-1 | Suntech Power STP285-VRM-1.5 | Suntech Power PLUTO290-Vdm | Suntech Power PLUTO290-Vdx | Suntech Power STP290-24-Vd | Suntech Power STP290-24-Vdx | Suntech Power STP290-24-Ve | Suntech Power STP290-VRM-1 | Suntech Power STP290-VRM-1.5 | Suntech Power PLUTO295-Vdm | Suntech Power PLUTO295-Vdx | Suntech Power STP295-24-Vd | Suntech Power STP295-24-Vdx | Suntech Power STP295-24-Ve | Suntech Power STP295-VRM-1 | Suntech Power STP295-VRM-1.5 | Suntech Power PLUTO300-Vdm | Suntech Power PLUTO300-Vdx | Suntech Power STP300-24-Vd | Suntech Power STP300-24-Vdx | Suntech Power STP300-24-Ve | Suntech Power STP300-VRM-1 | Suntech Power STP300-VRM-1.5 | Suntech Power PLUTO305-Vdm | Suntech Power PLUTO305-Vdx | Suntech Power STP305-24-Vd | Suntech Power STP305-24-Vdx | Suntech Power STP305-24-Ve | Suntech Power STP305-VRM-1 | Suntech Power STP305-VRM-1.5 | Suntech Power PLUTO310-Vdm | Suntech Power PLUTO310-Vdx | Suntech Power STP310-24-Vd | Suntech Power STP310-24-Vdx | Suntech Power STP310-24-Ve | Suntech Power STP310-VRM-1 | Suntech Power STP310-VRM-1.5 | Suntech Power STP315-24-Vd | Suntech Power STP315-24-Vdx | Suntech Power STP315-24-Ve | Suntech Power STP320-24-Vd | Suntech Power STP320-24-Vdx | Suntech Power STP320-24-Ve | Suntop Solar Energy TOP-S-125M6A | Suntop Solar Energy TOP-S-130M6A | Suntop Solar Energy TOP-S-135M6A | Suntop Solar Energy TOP-S-135S6A | Suntop Solar Energy TOP-S-140M6A | Suntop Solar Energy TOP-S-140S6A | Suntop Solar Energy TOP-S-145S6A | Suntop Solar Energy TOP-S-170M6A | Suntop Solar Energy TOP-S-175M6A | Suntop Solar Energy TOP-S-180M6A | Suntop Solar Energy TOP-S-185M6A | Suntop Solar Energy TOP-S-185S6A | Suntop Solar Energy TOP-S-190M6A | Suntop Solar Energy TOP-S-190S6A | Suntop Solar Energy TOP-S-195M6A | Suntop Solar Energy TOP-S-195S6A | Suntop Solar Energy TOP-S-200M6A | Suntop Solar Energy TOP-S-205M6A | Suntop Solar Energy TOP-S-210M6A | Suntop Solar Energy TOP-H-215M6A | Suntop Solar Energy TOP-S-215M6A | Suntop Solar Energy TOP-H-220M6A | Suntop Solar Energy TOP-H-220S6A | Suntop Solar Energy TOP-S-220M6A | Suntop Solar Energy TOP-S-220S6A | Suntop Solar Energy TOP-H-225M6A | Suntop Solar Energy TOP-H-225S6A | Suntop Solar Energy TOP-S-225M6A | Suntop Solar Energy TOP-S-225S6A | Suntop Solar Energy TOP-H-230M6A | Suntop Solar Energy TOP-H-230S6A | Suntop Solar Energy TOP-S-230M6A | Suntop Solar Energy TOP-S-230S6A | Suntop Solar Energy TOP-H-235M6A | Suntop Solar Energy TOP-H-235S6A | Suntop Solar Energy TOP-S-235M6A | Suntop Solar Energy TOP-S-235S6A | Suntop Solar Energy TOP-H-240S6A | Suntop Solar Energy TOP-S-240S6A | SunWize Technologies SW170 | SunWize Technologies SW175 | SunWize Technologies SW180 | Supreme Solar SS-165M | Supreme Solar SS-170M | Supreme Solar SS-175M | Supreme Solar SS-180M | Supreme Solar SS-200P | Supreme Solar SS-210P | Supreme Solar SS-220P | Supreme Solar SS-230P | Supreme Solar SS-240P | Supreme Solar SS-250P | Supreme Solar SS-260P | Supreme Solar SS-270P | Supreme Solar SS-280P | Suzhou Shenglong PV-Tech SLSM-175D | Suzhou Shenglong PV-Tech SLSM-180D | Suzhou Shenglong PV-Tech SLSM-185D | Suzhou Shenglong PV-Tech SLSM-220P | Suzhou Shenglong PV-Tech SLSM-225P | Suzhou Shenglong PV-Tech SLSM-230P | SweModule 220 x | SweModule 225 x | SweModule 230 x | SweModule 235 x | SweModule 240 x | SweModule 245 x | SweModule 250 x | SweModule 255 x | SweModule 260 x | SweModule 265 x | T & Solar TSS3-228 | T & Solar TSS3-230 | T & Solar TSS3-233 | T & Solar TSS3-235 | T & Solar TSS3-238 | T & Solar TSS3-240 | T & Solar TSS3-243 | T & Solar TSS3-245 | T & Solar TSS3-248 | T & Solar TSS3-250 | Tainergy Tech TKSE-13001 | Tainergy Tech TKSE-13501 | Tainergy Tech TKSE-14001 | Tainergy Tech TKSE-14501 | Tainergy Tech TKSD-15001 | Tainergy Tech TKSD-15501 | Tainergy Tech TKSD-16001 | Tainergy Tech TKSD-16501 | Tainergy Tech TKSC-17001 | Tainergy Tech TKSD-17001 | Tainergy Tech TKSC-17501 | Tainergy Tech TKSC-18001 | Tainergy Tech TKSC-18501 | Tainergy Tech TKSC-19001 | Tainergy Tech TKSC-19501 | Tainergy Tech TKSB-20001 | Tainergy Tech TKSB-20501 | Tainergy Tech TKSB-21001 | Tainergy Tech TKSB-21501 | Tainergy Tech TKSA-22001 | Tainergy Tech TKSB-22001 | Tainergy Tech TKSA-22501 | Tainergy Tech TKSA-23001 | Tainergy Tech TKSA-23501 | Tainergy Tech TKSA-24001 | Tainergy Tech TKSA-24501 | Tainergy Tech TKSA-25001 | Tainergy Tech TKSG-25001 | Tainergy Tech TKSA-25501 | Tainergy Tech TKSG-25501 | Tainergy Tech TKSA-26001 | Tainergy Tech TKSG-26001 | Tainergy Tech TKSG-26501 | Tainergy Tech TKSG-27001 | Tainergy Tech TKSG-27501 | Tainergy Tech TKSG-28001 | Tainergy Tech TKSG-28501 | Tainergy Tech TKSG-29001 | Tainergy Tech TKSG-29501 | Tainergy Tech TKSG-30001 | Tainergy Tech TKSG-30501 | Tainergy Tech TKSG-31001 | Tainergy Tech TKSG-31501 | Taiwan Semiconductor Manufacturing TS-230P4-AD | Taiwan Semiconductor Manufacturing TS-235P4-AD | Taiwan Semiconductor Manufacturing TS-240P4-AD | Taiwan Semiconductor Manufacturing TS-245P4-AD | Taiwan Semiconductor Manufacturing TS-250P4-AD | Talesun Solar TP660AM225 | Talesun Solar TP660AM240 | Tata Power Solar Systems TP140SBZ | Tata Power Solar Systems TP145SBZ | Tata Power Solar Systems TP150SBZ | Tata Power Solar Systems TP235MBZ | Tata Power Solar Systems TP240MBZ | Tata Power Solar Systems TP245MBZ | Tata Power Solar Systems TP250MBZ | Tata Power Solar Systems TP255MBZ | Tata Power Solar Systems TP265LBZ | Tata Power Solar Systems TP270LBZ | Tata Power Solar Systems TP275LBZ | Tata Power Solar Systems TP280LBZ | Tata Power Solar Systems TP285LBZ | Tata Power Solar Systems TP290LBZ | Tata Power Solar Systems TP295LBZ | Tata Power Solar Systems TP300LBZ | Tata Power Solar Systems TP305LBZ | Tata Power Solar Systems TP310LBZ | TBEA Xinjiang SunOasis TBEA4180T | TBEA Xinjiang SunOasis TBEA4185T | TBEA Xinjiang SunOasis TBEA4190T | TBEA Xinjiang SunOasis TBEA3220T | TBEA Xinjiang SunOasis TBEA3225T | TBEA Xinjiang SunOasis TBEA3230T | TBEA Xinjiang SunOasis TBEA3235T | TBEA Xinjiang SunOasis TBEA3240T | TDG Holding T170M725 | TDG Holding T175M725 | TDG Holding T180M725 | TDG Holding T185M725 | TDG Holding T190M725 | TDG Holding T195M725 | TDG Holding T200M725 | TDG Holding T210P606 | TDG Holding T215P606 | TDG Holding T220M606 | TDG Holding T220M965 | TDG Holding T220P606 | TDG Holding T225M606 | TDG Holding T225M965 | TDG Holding T225P606 | TDG Holding T230M606 | TDG Holding T230M965 | TDG Holding T230P606 | TDG Holding T235M606 | TDG Holding T235M965 | TDG Holding T235P606 | TDG Holding T240M606 | TDG Holding T240M965 | TDG Holding T240P606 | TDG Holding T245M606 | TDG Holding T245M965 | TDG Holding T245P606 | TDG Holding T250M606 | TDG Holding T250M965 | TDG Holding T250P606 | TDG Holding T250P726 | TDG Holding T255M606 | TDG Holding T255M726 | TDG Holding T255M965 | TDG Holding T255P726 | TDG Holding T260M726 | TDG Holding T260M965 | TDG Holding T260P726 | TDG Holding T265M726 | TDG Holding T265P726 | TDG Holding T270M726 | TDG Holding T270P726 | TDG Holding T275M726 | TDG Holding T275P726 | TDG Holding T280M726 | TDG Holding T280P726 | TDG Holding T285M726 | TDG Holding T285P726 | TDG Holding T290M726 | TDG Holding T290P726 | TDG Holding T295M726 | TDG Holding T295P726 | TDG Holding T300M726 | TDG Holding T305M726 | Tianwei Ecosolargy TWES-(155)72M | Tianwei Ecosolargy TWES-(160)72M | Tianwei Ecosolargy TWES-(165)72M | Tianwei Ecosolargy TWES-(170)72M | Tianwei Ecosolargy TWES-(175)72M | Tianwei Ecosolargy TWES-(180)72M | Tianwei Ecosolargy TWES-(200)60P | Tianwei Ecosolargy TWES-(205)60P | Tianwei Ecosolargy TWES-(210)60P | Tianwei Ecosolargy TWES-(215)60P | Tianwei Ecosolargy TWES-(220)60P | Tianwei Ecosolargy TWES-(225)60P | Tianwei Ecosolargy TWES-(230)60P | Tianwei Ecosolargy TWES-(235)60P | Tianwei New Energy (Chengdu) PV Module TW155(35)D | Tianwei New Energy (Chengdu) PV Module TW160(35)D | Tianwei New Energy (Chengdu) PV Module TW165(35)D | Tianwei New Energy (Chengdu) PV Module TW170(35)D | Tianwei New Energy (Chengdu) PV Module TW175(35)D | Tianwei New Energy (Chengdu) PV Module TW180(28)P | Tianwei New Energy (Chengdu) PV Module TW180(35)D | Tianwei New Energy (Chengdu) PV Module TW185(28)P | Tianwei New Energy (Chengdu) PV Module TW185(35)D | Tianwei New Energy (Chengdu) PV Module TW190(28)P | Tianwei New Energy (Chengdu) PV Module TW195(28)P | Tianwei New Energy (Chengdu) PV Module TW200(28)P | Tianwei New Energy (Chengdu) PV Module TW205(28)P | Tianwei New Energy (Chengdu) PV Module TW210(28)P | Tianwei New Energy (Chengdu) PV Module TW215(28)P | Tianwei New Energy (Chengdu) PV Module TW220(28)P | Tianwei New Energy (Chengdu) PV Module TW225(28)P | Tianwei New Energy (Chengdu) PV Module TW230(28)P | Tianwei New Energy (Chengdu) PV Module TW235(28)P | Tianwei New Energy (Yangzhou) TW240P660 | Tianwei New Energy (Yangzhou) TW240P660(1000) | Tianwei New Energy (Yangzhou) TW245P660 | Tianwei New Energy (Yangzhou) TW245P660(1000) | Tianwei New Energy (Yangzhou) TW250M660 | Tianwei New Energy (Yangzhou) TW250M660(1000) | Tianwei New Energy (Yangzhou) TW250P660 | Tianwei New Energy (Yangzhou) TW250P660(1000) | Tianwei New Energy (Yangzhou) TW255M660 | Tianwei New Energy (Yangzhou) TW255M660(1000) | Tianwei New Energy (Yangzhou) TW255P660 | Tianwei New Energy (Yangzhou) TW255P660(1000) | Tianwei New Energy (Yangzhou) TW260M660 | Tianwei New Energy (Yangzhou) TW260M660(1000) | Tianwei New Energy (Yangzhou) TW260P660 | Tianwei New Energy (Yangzhou) TW260P660(1000) | Tianwei New Energy (Yangzhou) TW265M660 | Tianwei New Energy (Yangzhou) TW265M660(1000) | Tianwei New Energy (Yangzhou) TW270M660 | Tianwei New Energy (Yangzhou) TW270M660(1000) | Tianwei New Energy (Yangzhou) TW285P672 | Tianwei New Energy (Yangzhou) TW285P672(1000) | Tianwei New Energy (Yangzhou) TW290M672 | Tianwei New Energy (Yangzhou) TW290M672(1000) | Tianwei New Energy (Yangzhou) TW290P672 | Tianwei New Energy (Yangzhou) TW290P672(1000) | Tianwei New Energy (Yangzhou) TW295M672 | Tianwei New Energy (Yangzhou) TW295M672(1000) | Tianwei New Energy (Yangzhou) TW295P672 | Tianwei New Energy (Yangzhou) TW295P672(1000) | Tianwei New Energy (Yangzhou) TW300M672 | Tianwei New Energy (Yangzhou) TW300M672(1000) | Tianwei New Energy (Yangzhou) TW300P672 | Tianwei New Energy (Yangzhou) TW300P672(1000) | Tianwei New Energy (Yangzhou) TW305M672 | Tianwei New Energy (Yangzhou) TW305M672(1000) | Tianwei New Energy (Yangzhou) TW305P672 | Tianwei New Energy (Yangzhou) TW305P672(1000) | Tianwei New Energy (Yangzhou) TW310M672 | Tianwei New Energy (Yangzhou) TW310M672(1000) | Tianwei New Energy (Yangzhou) TW310P672 | Tianwei New Energy (Yangzhou) TW310P672(1000) | Tianwei New Energy (Yangzhou) TW315M672 | Tianwei New Energy (Yangzhou) TW315M672(1000) | Tianwei New Energy (Yangzhou) TW320M672 | Tianwei New Energy (Yangzhou) TW320M672(1000) | Tianwei New Energy Holdings TW210P60-FA2 | Tianwei New Energy Holdings TW215P60-FA2 | Tianwei New Energy Holdings TW220P60-FA2 | Tianwei New Energy Holdings TW225P60-FA2 | Tianwei New Energy Holdings TW230P60-FA2 | Tianwei New Energy Holdings TW235P60-FA2 | Tianwei New Energy Holdings TW240P60-FA2 | Titan Energy Systems Titan S6-60 | Titan Energy Systems Titan S6-60-2-235 | Titan Energy Systems Titan S6-60-2-240 | Titan Energy Systems Titan S6-60-2-245 | Top Solar TSC-200W-E | Topsun TS-M228NA1 | Topsun TS-M229NA1 | Topsun TS-M230NA1 | Topsun TS-M231NA1 | Topsun TS-M232NA1 | Topsun TS-M233NA1 | Topsun TS-M234NA1 | Topsun TS-M235NA1 | Topsun TS-M236NA1 | Topsun TS-M237NA1 | Topsun TS-M238NA1 | Topsun TS-S238SA1K | Topsun TS-S238TA1 | Topsun TS-M239NA1 | Topsun TS-S239SA1K | Topsun TS-S239TA1 | Topsun TS-M240NA1 | Topsun TS-S240SA1K | Topsun TS-S240TA1 | Topsun TS-M241NA1 | Topsun TS-S241SA1K | Topsun TS-S241TA1 | Topsun TS-M242NA1 | Topsun TS-S242SA1K | Topsun TS-S242TA1 | Topsun TS-M243NA1 | Topsun TS-S243SA1K | Topsun TS-S243TA1 | Topsun TS-M244NA1 | Topsun TS-S244SA1K | Topsun TS-S244TA1 | Topsun TS-M245NA1 | Topsun TS-S245SA1K | Topsun TS-S245TA1 | Topsun TS-M246NA1 | Topsun TS-S246SA1K | Topsun TS-S246TA1 | Topsun TS-M247NA1 | Topsun TS-S247SA1K | Topsun TS-S247TA1 | Topsun TS-M248NA1 | Topsun TS-S248SA1K | Topsun TS-S248TA1 | Topsun TS-M249NA1 | Topsun TS-S249SA1K | Topsun TS-S249TA1 | Topsun TS-M250NA1 | Topsun TS-S250SA1K | Topsun TS-S250TA1 | Topsun TS-M251NA1 | Topsun TS-S251SA1K | Topsun TS-S251TA1 | Topsun TS-M252NA1 | Topsun TS-S252SA1K | Topsun TS-S252TA1 | Topsun TS-S253SA1K | Topsun TS-S253TA1 | Topsun TS-S254SA1K | Topsun TS-S254TA1 | Topsun TS-S255SA1K | Topsun TS-S255TA1 | Topsun TS-S256SA1K | Topsun TS-S256TA1 | Topsun TS-S257SA1K | Topsun TS-S257TA1 | Topsun TS-S258SA1K | Topsun TS-S258TA1 | Topsun TS-S259SA1K | Topsun TS-S259TA1 | Topsun TS-S260SA1K | Topsun TS-S260TA1 | Topsun TS-S261SA1K | Topsun TS-S261TA1 | Topsun TS-S262SA1K | Topsun TS-S262TA1 | Topsun TS-S286SA1K | Topsun TS-S287SA1K | Topsun TS-S288SA1K | Topsun TS-S289SA1K | Topsun TS-S290SA1K | Topsun TS-S291SA1K | Topsun TS-S292SA1K | Topsun TS-S293SA1K | Topsun TS-S294SA1K | Topsun TS-S295SA1K | Topsun TS-S296SA1K | Topsun TS-S297SA1K | Topsun TS-S298SA1K | Topsun TS-S299SA1K | Topsun TS-S300SA1K | Topsun TS-S301SA1K | Topsun TS-S302SA1K | Topsun TS-S303SA1K | Topsun TS-S304SA1K | Topsun TS-S305SA1K | Topsun TS-S306SA1K | Topsun TS-S307SA1K | Topsun TS-S308SA1K | Topsun TS-S309SA1K | Topsun TS-S310SA1K | Topsun TS-S311SA1K | Topsun TS-S312SA1K | Topsun TS-S313SA1K | Topsun TS-S314SA1K | Topsun TS-S356TA1 | Topsun TS-S357TA1 | Topsun TS-S358TA1 | Topsun TS-S359TA1 | Topsun TS-S360TA1 | Topsun TS-M361NA1 | Topsun TS-S361TA1 | Topsun TS-M362NA1 | Topsun TS-S362TA1 | Topsun TS-M363NA1 | Topsun TS-S363TA1 | Topsun TS-M364NA1 | Topsun TS-S364TA1 | Topsun TS-M365NA1 | Topsun TS-S365TA1 | Topsun TS-M366NA1 | Topsun TS-S366TA1 | Topsun TS-M367NA1 | Topsun TS-S367TA1 | Topsun TS-M368NA1 | Topsun TS-S368TA1 | Topsun TS-M369NA1 | Topsun TS-S369TA1 | Topsun TS-M370NA1 | Topsun TS-S370 | Topsun TS-S370TA1 | Topsun TS-M371NA1 | Topsun TS-S371 | Topsun TS-S371TA1 | Topsun TS-M372NA1 | Topsun TS-S372 | Topsun TS-S372TA1 | Topsun TS-M373NA1 | Topsun TS-S373 | Topsun TS-S373TA1 | Topsun TS-M374NA1 | Topsun TS-S374 | Topsun TS-S374TA1 | Topsun TS-M375NA1 | Topsun TS-S375 | Topsun TS-S375TA1 | Topsun TS-M376NA1 | Topsun TS-S376 | Topsun TS-S376TA1 | Topsun TS-M377NA1 | Topsun TS-S377 | Topsun TS-S377TA1 | Topsun TS-M378NA1 | Topsun TS-S378 | Topsun TS-S378TA1 | Topsun TS-M379NA1 | Topsun TS-S379 | Topsun TS-S379TA1 | Topsun TS-M380NA1 | Topsun TS-S380 | Topsun TS-S380SA1 | Topsun TS-S380TA1 | Topsun TS-S380VA1 | Topsun TS-M381JA1 | Topsun TS-M381NA1 | Topsun TS-S381 | Topsun TS-S381SA1 | Topsun TS-S381SA1K | Topsun TS-S381TA1 | Topsun TS-S381VA1 | Topsun TS-M382JA1 | Topsun TS-M382NA1 | Topsun TS-S382 | Topsun TS-S382SA1 | Topsun TS-S382SA1K | Topsun TS-S382TA1 | Topsun TS-S382VA1 | Topsun TS-M383JA1 | Topsun TS-M383NA1 | Topsun TS-S383 | Topsun TS-S383SA1 | Topsun TS-S383SA1K | Topsun TS-S383TA1 | Topsun TS-S383VA1 | Topsun TS-M384JA1 | Topsun TS-M384NA1 | Topsun TS-S384 | Topsun TS-S384SA1 | Topsun TS-S384SA1K | Topsun TS-S384TA1 | Topsun TS-S384VA1 | Topsun TS-M385JA1 | Topsun TS-M385NA1 | Topsun TS-S385 | Topsun TS-S385SA1 | Topsun TS-S385SA1K | Topsun TS-S385TA1 | Topsun TS-S385VA1 | Topsun TS-M386JA1 | Topsun TS-M386NA1 | Topsun TS-S386 | Topsun TS-S386SA1 | Topsun TS-S386SA1K | Topsun TS-S386TA1 | Topsun TS-S386VA1 | Topsun TS-M387JA1 | Topsun TS-M387NA1 | Topsun TS-S387 | Topsun TS-S387SA1 | Topsun TS-S387SA1K | Topsun TS-S387TA1 | Topsun TS-S387VA1 | Topsun TS-M388JA1 | Topsun TS-M388NA1 | Topsun TS-S388 | Topsun TS-S388SA1 | Topsun TS-S388SA1K | Topsun TS-S388TA1 | Topsun TS-S388VA1 | Topsun TS-M389JA1 | Topsun TS-M389NA1 | Topsun TS-S389 | Topsun TS-S389SA1 | Topsun TS-S389SA1K | Topsun TS-S389TA1 | Topsun TS-S389VA1 | Topsun TS-M390JA1 | Topsun TS-M390NA1 | Topsun TS-S390 | Topsun TS-S390SA1 | Topsun TS-S390SA1K | Topsun TS-S390TA1 | Topsun TS-S390VA1 | Topsun TS-M391JA1 | Topsun TS-M391NA1 | Topsun TS-S391 | Topsun TS-S391SA1 | Topsun TS-S391SA1K | Topsun TS-S391TA1 | Topsun TS-S391VA1 | Topsun TS-M392JA1 | Topsun TS-M392NA1 | Topsun TS-S392 | Topsun TS-S392SA1 | Topsun TS-S392SA1K | Topsun TS-S392TA1 | Topsun TS-S392VA1 | Topsun TS-M393JA1 | Topsun TS-M393NA1 | Topsun TS-S393 | Topsun TS-S393SA1 | Topsun TS-S393SA1K | Topsun TS-S393TA1 | Topsun TS-S393VA1 | Topsun TS-M394JA1 | Topsun TS-M394NA1 | Topsun TS-S394 | Topsun TS-S394SA1 | Topsun TS-S394SA1K | Topsun TS-S394TA1 | Topsun TS-S394VA1 | Topsun TS-M395JA1 | Topsun TS-M395NA1 | Topsun TS-S395 | Topsun TS-S395SA1 | Topsun TS-S395SA1K | Topsun TS-S395TA1 | Topsun TS-S395VA1 | Topsun TS-M396JA1 | Topsun TS-M396NA1 | Topsun TS-S396 | Topsun TS-S396SA1 | Topsun TS-S396SA1K | Topsun TS-S396TA1 | Topsun TS-S396VA1 | Topsun TS-M397JA1 | Topsun TS-M397NA1 | Topsun TS-S397 | Topsun TS-S397SA1 | Topsun TS-S397SA1K | Topsun TS-S397TA1 | Topsun TS-S397VA1 | Topsun TS-M398JA1 | Topsun TS-M398NA1 | Topsun TS-S398 | Topsun TS-S398SA1 | Topsun TS-S398SA1K | Topsun TS-S398TA1 | Topsun TS-S398VA1 | Topsun TS-M399JA1 | Topsun TS-M399NA1 | Topsun TS-S399 | Topsun TS-S399SA1 | Topsun TS-S399SA1K | Topsun TS-S399TA1 | Topsun TS-S399VA1 | Topsun TS-M400JA1 | Topsun TS-S400 | Topsun TS-S400SA1 | Topsun TS-S400SA1K | Topsun TS-S400TA1 | Topsun TS-S400VA1 | Topsun TS-M401JA1 | Topsun TS-S401 | Topsun TS-S401SA1 | Topsun TS-S401SA1K | Topsun TS-S401TA1 | Topsun TS-S401VA1 | Topsun TS-M402JA1 | Topsun TS-S402 | Topsun TS-S402SA1 | Topsun TS-S402SA1K | Topsun TS-S402TA1 | Topsun TS-S402VA1 | Topsun TS-M403JA1 | Topsun TS-S403 | Topsun TS-S403SA1 | Topsun TS-S403SA1K | Topsun TS-S403TA1 | Topsun TS-S403VA1 | Topsun TS-M404JA1 | Topsun TS-S404 | Topsun TS-S404SA1 | Topsun TS-S404SA1K | Topsun TS-S404TA1 | Topsun TS-S404VA1 | Topsun TS-M405JA1 | Topsun TS-S405 | Topsun TS-S405SA1 | Topsun TS-S405SA1K | Topsun TS-S405TA1 | Topsun TS-S405VA1 | Topsun TS-M406JA1 | Topsun TS-S406 | Topsun TS-S406SA1 | Topsun TS-S406SA1K | Topsun TS-S406TA1 | Topsun TS-S406VA1 | Topsun TS-M407JA1 | Topsun TS-S407 | Topsun TS-S407SA1 | Topsun TS-S407SA1K | Topsun TS-S407TA1 | Topsun TS-S407VA1 | Topsun TS-M408JA1 | Topsun TS-S408 | Topsun TS-S408SA1 | Topsun TS-S408SA1K | Topsun TS-S408TA1 | Topsun TS-S408VA1 | Topsun TS-M409JA1 | Topsun TS-S409 | Topsun TS-S409SA1 | Topsun TS-S409SA1K | Topsun TS-S409TA1 | Topsun TS-S409VA1 | Topsun TS-M410JA1 | Topsun TS-S410 | Topsun TS-S410SA1 | Topsun TS-S410SA1K | Topsun TS-S410TA1 | Topsun TS-S410VA1 | Topsun TS-M411JA1 | Topsun TS-S411SA1 | Topsun TS-S411SA1K | Topsun TS-S411TA1 | Topsun TS-S411VA1 | Topsun TS-M412JA1 | Topsun TS-S412SA1 | Topsun TS-S412SA1K | Topsun TS-S412TA1 | Topsun TS-S412VA1 | Topsun TS-M413JA1 | Topsun TS-S413SA1 | Topsun TS-S413SA1K | Topsun TS-S413TA1 | Topsun TS-S413VA1 | Topsun TS-M414JA1 | Topsun TS-S414SA1 | Topsun TS-S414SA1K | Topsun TS-S414TA1 | Topsun TS-S414VA1 | Topsun TS-M415JA1 | Topsun TS-S415SA1 | Topsun TS-S415SA1K | Topsun TS-S415TA1 | Topsun TS-S415VA1 | Topsun TS-M416JA1 | Topsun TS-S416SA1 | Topsun TS-S416SA1K | Topsun TS-S416TA1 | Topsun TS-S416VA1 | Topsun TS-M417JA1 | Topsun TS-S417SA1 | Topsun TS-S417SA1K | Topsun TS-S417TA1 | Topsun TS-S417VA1 | Topsun TS-M418JA1 | Topsun TS-S418SA1 | Topsun TS-S418SA1K | Topsun TS-S418TA1 | Topsun TS-S418VA1 | Topsun TS-M419JA1 | Topsun TS-S419SA1 | Topsun TS-S419SA1K | Topsun TS-S419TA1 | Topsun TS-M420JA1 | Topsun TS-S420SA1 | Topsun TS-S420TA1 | Trina Solar TSM-165DA01 | Trina Solar TSM-170D | Trina Solar TSM-170DA01 | Trina Solar TSM-170DA03 | Trina Solar TSM-170PA03 | Trina Solar TSM-175D | Trina Solar TSM-175DA01 | Trina Solar TSM-175DA03 | Trina Solar TSM-175PA03 | Trina Solar TSM-180D | Trina Solar TSM-180DA01 | Trina Solar TSM-180DA03 | Trina Solar TSM-180PA03 | Trina Solar TSM-185DA01 | Trina Solar TSM-185DA01A | Trina Solar TSM-185DA01A.05 | Trina Solar TSM-185DA01A.08 | Trina Solar TSM-185DA03 | Trina Solar TSM-185PA03 | Trina Solar TSM-190DA01A | Trina Solar TSM-190DA01A.05 | Trina Solar TSM-190DA01A.08 | Trina Solar TSM-190DA03 | Trina Solar TSM-190PA03 | Trina Solar TSM-195DA01A | Trina Solar TSM-195DA01A.05 | Trina Solar TSM-195DA01A.08 | Trina Solar TSM-200DA01A | Trina Solar TSM-200DA01A.05 | Trina Solar TSM-200DA01A.08 | Trina Solar TSM-205DA01A | Trina Solar TSM-205DA01A.05 | Trina Solar TSM-205DA01A.08 | Trina Solar TSM-220DA05 | Trina Solar TSM-220PA05 | Trina Solar TSM-220PA05.05 | Trina Solar TSM-220PA05.08 | Trina Solar TSM-220PA05.10 | Trina Solar TSM-220PA05.15 | Trina Solar TSM-220PA05.18 | Trina Solar TSM-220PA05.20 | Trina Solar TSM-220PA05.28 | Trina Solar TSM-220PA05.30 | Trina Solar TSM-220PA05.38 | Trina Solar TSM-220PD05 | Trina Solar TSM-220PD05.08 | Trina Solar TSM-220PD05.10 | Trina Solar TSM-220PD05.18 | Trina Solar TSM-225PA05 | Trina Solar TSM-225PA05.05 | Trina Solar TSM-225PA05.08 | Trina Solar TSM-225PA05.10 | Trina Solar TSM-225PA05.15 | Trina Solar TSM-225PA05.18 | Trina Solar TSM-225PA05.20 | Trina Solar TSM-225PA05.28 | Trina Solar TSM-225PA05.30 | Trina Solar TSM-225PA05.38 | Trina Solar TSM-225PD05 | Trina Solar TSM-225PD05.08 | Trina Solar TSM-225PD05.10 | Trina Solar TSM-225PD05.18 | Trina Solar TSM-230DA05 | Trina Solar TSM-230PA05 | Trina Solar TSM-230PA05.05 | Trina Solar TSM-230PA05.08 | Trina Solar TSM-230PA05.10 | Trina Solar TSM-230PA05.15 | Trina Solar TSM-230PA05.18 | Trina Solar TSM-230PA05.20 | Trina Solar TSM-230PA05.28 | Trina Solar TSM-230PA05.30 | Trina Solar TSM-230PA05.38 | Trina Solar TSM-230PD05 | Trina Solar TSM-230PD05.08 | Trina Solar TSM-230PD05.10 | Trina Solar TSM-230PD05.18 | Trina Solar TSM-235PA05 | Trina Solar TSM-235PA05.05 | Trina Solar TSM-235PA05.08 | Trina Solar TSM-235PA05.10 | Trina Solar TSM-235PA05.15 | Trina Solar TSM-235PA05.18 | Trina Solar TSM-235PA05.20 | Trina Solar TSM-235PA05.28 | Trina Solar TSM-235PA05.30 | Trina Solar TSM-235PA05.38 | Trina Solar TSM-235PD05 | Trina Solar TSM-235PD05.08 | Trina Solar TSM-235PD05.10 | Trina Solar TSM-235PD05.18 | Trina Solar TSM-240DA05 | Trina Solar TSM-240PA05 | Trina Solar TSM-240PA05.05 | Trina Solar TSM-240PA05.08 | Trina Solar TSM-240PA05.10 | Trina Solar TSM-240PA05.15 | Trina Solar TSM-240PA05.18 | Trina Solar TSM-240PA05.20 | Trina Solar TSM-240PA05.28 | Trina Solar TSM-240PA05.30 | Trina Solar TSM-240PA05.38 | Trina Solar TSM-240PD05 | Trina Solar TSM-240PD05.08 | Trina Solar TSM-240PD05.10 | Trina Solar TSM-240PD05.18 | Trina Solar TSM-240PDG5 | Trina Solar TSM-240PDG5.50 | Trina Solar TSM-245PA05 | Trina Solar TSM-245PA05.05 | Trina Solar TSM-245PA05.08 | Trina Solar TSM-245PA05.10 | Trina Solar TSM-245PA05.15 | Trina Solar TSM-245PA05.18 | Trina Solar TSM-245PA05.20 | Trina Solar TSM-245PA05.28 | Trina Solar TSM-245PA05.30 | Trina Solar TSM-245PA05.38 | Trina Solar TSM-245PD05 | Trina Solar TSM-245PD05.08 | Trina Solar TSM-245PD05.10 | Trina Solar TSM-245PD05.18 | Trina Solar TSM-245PDG5 | Trina Solar TSM-245PDG5.50 | Trina Solar TSM-250PA05 | Trina Solar TSM-250PA05.05 | Trina Solar TSM-250PA05.08 | Trina Solar TSM-250PA05.10 | Trina Solar TSM-250PA05.15 | Trina Solar TSM-250PA05.18 | Trina Solar TSM-250PA05.20 | Trina Solar TSM-250PA05.28 | Trina Solar TSM-250PA05.30 | Trina Solar TSM-250PA05.38 | Trina Solar TSM-250PA05A | Trina Solar TSM-250PA05A.08 | Trina Solar TSM-250PA05A.10 | Trina Solar TSM-250PA05A.18 | Trina Solar TSM-250PD05 | Trina Solar TSM-250PD05.08 | Trina Solar TSM-250PD05.10 | Trina Solar TSM-250PD05.18 | Trina Solar TSM-250PDG5 | Trina Solar TSM-250PDG5.50 | Trina Solar TSM-255PA05 | Trina Solar TSM-255PA05.08 | Trina Solar TSM-255PA05.10 | Trina Solar TSM-255PA05.18 | Trina Solar TSM-255PA05.20 | Trina Solar TSM-255PA05.28 | Trina Solar TSM-255PA05.30 | Trina Solar TSM-255PA05.38 | Trina Solar TSM-255PA05A | Trina Solar TSM-255PA05A.08 | Trina Solar TSM-255PA05A.10 | Trina Solar TSM-255PA05A.18 | Trina Solar TSM-255PD05 | Trina Solar TSM-255PD05.08 | Trina Solar TSM-255PD05.10 | Trina Solar TSM-255PD05.18 | Trina Solar TSM-255PDG5 | Trina Solar TSM-255PDG5.50 | Trina Solar TSM-260PA05 | Trina Solar TSM-260PA05.08 | Trina Solar TSM-260PA05.10 | Trina Solar TSM-260PA05.18 | Trina Solar TSM-260PA05.20 | Trina Solar TSM-260PA05.28 | Trina Solar TSM-260PA05.30 | Trina Solar TSM-260PA05.38 | Trina Solar TSM-260PA05A | Trina Solar TSM-260PA05A.08 | Trina Solar TSM-260PA05A.10 | Trina Solar TSM-260PA05A.18 | Trina Solar TSM-260PD05 | Trina Solar TSM-260PD05.08 | Trina Solar TSM-260PD05.10 | Trina Solar TSM-260PD05.18 | Trina Solar TSM-260PDG5 | Trina Solar TSM-260PDG5.50 | Trina Solar TSM-265PA05A | Trina Solar TSM-265PA05A.08 | Trina Solar TSM-265PA05A.10 | Trina Solar TSM-265PA05A.18 | Trina Solar TSM-270PA05A | Trina Solar TSM-270PA05A.08 | Trina Solar TSM-270PA05A.10 | Trina Solar TSM-270PA05A.18 | Trina Solar TSM-270PA14 | Trina Solar TSM-270PA14.05 | Trina Solar TSM-270PA14.08 | Trina Solar TSM-270PA14.10 | Trina Solar TSM-270PA14.18 | Trina Solar TSM-270PA14.20 | Trina Solar TSM-270PA14.28 | Trina Solar TSM-270PD14.08 | Trina Solar TSM-270PD14.10 | Trina Solar TSM-270PD14.18 | Trina Solar TSM-275PA14 | Trina Solar TSM-275PA14.05 | Trina Solar TSM-275PA14.08 | Trina Solar TSM-275PA14.10 | Trina Solar TSM-275PA14.18 | Trina Solar TSM-275PA14.20 | Trina Solar TSM-275PA14.28 | Trina Solar TSM-275PD14 | Trina Solar TSM-275PD14.08 | Trina Solar TSM-275PD14.10 | Trina Solar TSM-275PD14.18 | Trina Solar TSM-280PA14 | Trina Solar TSM-280PA14.05 | Trina Solar TSM-280PA14.08 | Trina Solar TSM-280PA14.10 | Trina Solar TSM-280PA14.18 | Trina Solar TSM-280PA14.20 | Trina Solar TSM-280PA14.28 | Trina Solar TSM-280PD14 | Trina Solar TSM-280PD14.08 | Trina Solar TSM-280PD14.10 | Trina Solar TSM-280PD14.18 | Trina Solar TSM-285PA14 | Trina Solar TSM-285PA14.05 | Trina Solar TSM-285PA14.08 | Trina Solar TSM-285PA14.10 | Trina Solar TSM-285PA14.18 | Trina Solar TSM-285PA14.20 | Trina Solar TSM-285PA14.28 | Trina Solar TSM-285PA14A | Trina Solar TSM-285PA14A.08 | Trina Solar TSM-285PD14 | Trina Solar TSM-285PD14.08 | Trina Solar TSM-285PD14.10 | Trina Solar TSM-285PD14.18 | Trina Solar TSM-290PA14 | Trina Solar TSM-290PA14.08 | Trina Solar TSM-290PA14.10 | Trina Solar TSM-290PA14.18 | Trina Solar TSM-290PA14.20 | Trina Solar TSM-290PA14.28 | Trina Solar TSM-290PA14A | Trina Solar TSM-290PA14A.08 | Trina Solar TSM-290PD14 | Trina Solar TSM-290PD14.08 | Trina Solar TSM-290PD14.10 | Trina Solar TSM-290PD14.18 | Trina Solar TSM-295PA14 | Trina Solar TSM-295PA14.08 | Trina Solar TSM-295PA14.10 | Trina Solar TSM-295PA14.18 | Trina Solar TSM-295PA14.20 | Trina Solar TSM-295PA14.28 | Trina Solar TSM-295PA14A | Trina Solar TSM-295PA14A.08 | Trina Solar TSM-295PD14 | Trina Solar TSM-295PD14.08 | Trina Solar TSM-295PD14.10 | Trina Solar TSM-295PD14.18 | Trina Solar TSM-300PA14 | Trina Solar TSM-300PA14.08 | Trina Solar TSM-300PA14.10 | Trina Solar TSM-300PA14.18 | Trina Solar TSM-300PA14.20 | Trina Solar TSM-300PA14.28 | Trina Solar TSM-300PA14A | Trina Solar TSM-300PA14A.08 | Trina Solar TSM-300PD14 | Trina Solar TSM-300PD14.08 | Trina Solar TSM-300PD14.10 | Trina Solar TSM-300PD14.18 | Trina Solar TSM-305PA14 | Trina Solar TSM-305PA14.08 | Trina Solar TSM-305PA14.10 | Trina Solar TSM-305PA14.18 | Trina Solar TSM-305PA14.20 | Trina Solar TSM-305PA14.28 | Trina Solar TSM-305PA14A | Trina Solar TSM-305PA14A.08 | Trina Solar TSM-305PD14 | Trina Solar TSM-305PD14.08 | Trina Solar TSM-305PD14.10 | Trina Solar TSM-305PD14.18 | Trina Solar TSM-310PA14 | Trina Solar TSM-310PA14.08 | Trina Solar TSM-310PA14.10 | Trina Solar TSM-310PA14.18 | Trina Solar TSM-310PA14.20 | Trina Solar TSM-310PA14.28 | Trina Solar TSM-310PA14A | Trina Solar TSM-310PA14A.08 | Trina Solar TSM-310PD14 | Trina Solar TSM-310PD14.08 | Trina Solar TSM-310PD14.10 | Trina Solar TSM-310PD14.18 | Trina Solar TSM-315PA14A | Trina Solar TSM-315PA14A.08 | TSEC TS36-6P2-130 | TSEC TS36-6M2-135 | TSEC TS36-6P2-135 | TSEC TS36-6M2-140 | TSEC TS36-6P2-140 | TSEC TS36-6M2-145 | TSEC TS48-6P2-175 | TSEC TS48-6M2-180 | TSEC TS48-6P2-180 | TSEC TS48-6M2-185 | TSEC TS48-6P2-185 | TSEC TS48-6M2-190 | TSEC TS54-6P2-190 | TSEC TS54-6M2-195 | TSEC TS54-6P2-195 | TSEC TS54-6M2-200 | TSEC TS54-6P2-200 | TSEC TS54-6M2-205 | TSEC TS54-6P2-205 | TSEC TS54-6M2-210 | TSEC TS54-6P2-210 | TSEC TS54-6M2-215 | TSEC TS54-6P2-215 | TSEC TS54-6M2-220 | TSEC TS60-6P2-220 | TSEC TS60-6M2-225 | TSEC TS60-6P2-225 | TSEC TS60-6M2-230 | TSEC TS60-6P2-230 | TSEC TS60-6M2-235 | TSEC TS60-6P2-235 | TSEC TS60-6M2-240 | TSEC TS60-6P2-240 | TSEC TS72-6P3-270 | TSEC TS72-6P2-275 | TSEC TS72-6P3-275 | TSEC TS72-6P2-280 | TSEC TS72-6P3-280 | TSEC TS72-6M3-285 | TSEC TS72-6P2-285 | TSEC TS72-6P3-285 | TSEC TS72-6M3-290 | TSEC TS72-6P2-290 | TSEC TS72-6P3-290 | TSEC TS72-6M3-295 | TSEC TS72-6P2-295 | TSEC TS72-6M3-300 | TSEC TS72-6M3-305 | TSMC Solar TS-110C | TSMC Solar TS-115C | TSMC Solar TS-120C | TSMC Solar TS-125C | TSMC Solar TS-130C | TSMC Solar TS-135C | TSMC Solar TS-135C1 | TSMC Solar TS-135C2 | TSMC Solar TS-140C1 | TSMC Solar TS-140C2 | TSMC Solar TS-145C1 | TSMC Solar TS-145C2 | TSMC Solar TS-150C1 | TSMC Solar TS-150C2 | TSMC Solar TS-155C1 | TSMC Solar TS-155C2 | TSMC Solar TS-160C1 | T-Solar Global TS102 | T-Solar Global TS370 | T-Solar Global TS390 | T-Solar Global TS410 | T-Solar Global TS92 | T-Solar Global TS97 | Tynsolar TYNS62409130 | Tynsolar TYNS62606130 | Tynsolar TYNS62409135 | Tynsolar TYNS62606135 | Tynsolar TYNS62409140 | Tynsolar TYNS62606140 | Tynsolar TYNS62409145 | Tynsolar TYNS62606145 | Tynsolar TYNS62607145 | Tynsolar TYNS62409150 | Tynsolar TYNS62606150 | Tynsolar TYNS62607150 | Tynsolar TYNS62409155 | Tynsolar TYNS62606155 | Tynsolar TYNS62607155 | Tynsolar TYNS62607160 | Tynsolar TYNS62608160 | TynSolar TYN-168P6 | Tynsolar TYNS62607165 | Tynsolar TYNS62608165 | TynSolar TYN-170S5 | Tynsolar TYNS62607170 | Tynsolar TYNS62608170 | TynSolar TYN-180P6 | TynSolar TYN-180S5 | Tynsolar TYNS62607175 | Tynsolar TYNS62608175 | Tynsolar TYNS62607180 | Tynsolar TYNS62608180 | Tynsolar TYNS62608185 | TynSolar TYN-190P6 | Tynsolar TYNS62608190 | TynSolar TYN-195P6 | Tynsolar TYNS62608195 | Tynsolar TYNS62609195 | TynSolar TYN-200P6 | Tynsolar TYNS62608200 | Tynsolar TYNS62609200 | TynSolar TYN-205P6 | Tynsolar TYNS62608205 | Tynsolar TYNS62609205 | TynSolar TYN-210P6 | Tynsolar TYNP62610210 | Tynsolar TYNS62608210 | Tynsolar TYNS62609210 | TynSolar TYN-215P6 | Tynsolar TYNP62610215 | Tynsolar TYNS62609215 | TynSolar TYN-220P6 | Tynsolar TYNP62610220 | Tynsolar TYNS62609220 | TynSolar TYN-225P6 | Tynsolar TYNP62610225 | Tynsolar TYNS62609225 | Tynsolar TYNS62610225 | TynSolar TYN-230P6 | Tynsolar TYNP62610230 | Tynsolar TYNS62609230 | Tynsolar TYNS62610230 | TynSolar TYN-235P6 | Tynsolar TYNP62610235 | Tynsolar TYNS62609235 | Tynsolar TYNS62610235 | TynSolar TYN-240P6 | Tynsolar TYNP62610240 | Tynsolar TYNP62611240 | Tynsolar TYNP62611250 | Tynsolar TYNS62610240 | TynSolar TYN-245P6 | Tynsolar TYNP62610245 | Tynsolar TYNP62611245 | Tynsolar TYNS62610245 | TynSolar TYN-250P6 | Tynsolar TYNP62610250 | Tynsolar TYNS62610250 | Tynsolar TYNS62611250 | TynSolar TYN-255P6 | Tynsolar TYNP62610255 | Tynsolar TYNP62611255 | Tynsolar TYNP62612255 | Tynsolar TYNS62610255 | Tynsolar TYNS62611255 | TynSolar TYN-260P6 | Tynsolar TYNP62611260 | Tynsolar TYNP62612260 | Tynsolar TYNS62610260 | Tynsolar TYNS62611260 | TynSolar TYN-265P6 | Tynsolar TYNP62611265 | Tynsolar TYNP62612265 | Tynsolar TYNS62611265 | Tynsolar TYNS62612265 | TynSolar TYN-270P6 | Tynsolar TYNP62611270 | Tynsolar TYNP62612270 | Tynsolar TYNS62611270 | Tynsolar TYNS62612270 | TynSolar TYN-275P6 | Tynsolar TYNP62611275 | Tynsolar TYNP62612275 | Tynsolar TYNS62611275 | Tynsolar TYNS62612275 | TynSolar TYN-280P6 | Tynsolar TYNP62611280 | Tynsolar TYNP62612280 | Tynsolar TYNS62611280 | Tynsolar TYNS62612280 | TynSolar TYN-285P6 | Tynsolar TYNP62612285 | Tynsolar TYNS62611285 | Tynsolar TYNS62612285 | Tynsolar TYNP62612290 | Tynsolar TYNS62612290 | Tynsolar TYNP62612295 | Tynsolar TYNS62612295 | Tynsolar TYNP62612300 | Tynsolar TYNS62612300 | Tynsolar TYNP62612305 | Tynsolar TYNS62612305 | Tynsolar TYNP62612310 | Tynsolar TYNS62612310 | Tynsolar TYNP62612315 | Tynsolar TYNS62612315 | U.S. Yabang Solar Energy CSM-220P | U.S. Yabang Solar Energy CSM-230P | U.S. Yabang Solar Energy CSM-235P | U.S. Yabang Solar Energy CSM-240PA | U.S. Yabang Solar Energy CSM-260P | U.S. Yabang Solar Energy CSM-270P | U.S. Yabang Solar Energy CSM-280P | U.S. Yabang Solar Energy CSM-290D-C | U.S. Yabang Solar Energy CSM-290P | U.S. Yabang Solar Energy CSM 295D-C | U.S. Yabang Solar Energy CSM-295P | U.S. Yabang Solar Energy CSM-300D-C | UE Solar ZHM175 | UE Solar ZHM180 | UE Solar ZHM185 | UE Solar ZHM220P | UE Solar ZHM225P | UE Solar ZHM230P | UE Solar ZHM235P | UE Solar ZHM240P | UE Solar ZHM245P | UE Solar ZHM250P | UE Solar ZHM255P | UE Solar ZHM260P | UE Solar ZHM265P | UE Solar ZHM270P | UE Solar ZHM275P | UE Solar ZHM280P | Unicor Federal Prison Industries PVM220PS-A2P1200 | Unicor Federal Prison Industries PVM220PS-G156200 | Unicor Federal Prison Industries PVM220PS-IM156200 | Unicor Federal Prison Industries PVM220PS-M156200 | Unicor Federal Prison Industries PVM220PS-Q6LTT200 | Unicor Federal Prison Industries PVM220PS-A2P1205 | Unicor Federal Prison Industries PVM220PS-G156205 | Unicor Federal Prison Industries PVM220PS-IM156205 | Unicor Federal Prison Industries PVM220PS-M156205 | Unicor Federal Prison Industries PVM220PS-Q6LTT205 | Unicor Federal Prison Industries PVM220PS-A2P1210 | Unicor Federal Prison Industries PVM220PS-G156210 | Unicor Federal Prison Industries PVM220PS-IM156210 | Unicor Federal Prison Industries PVM220PS-M156210 | Unicor Federal Prison Industries PVM220PS-Q6LTT210 | Unicor Federal Prison Industries PVM220PS-A2P1215 | Unicor Federal Prison Industries PVM220PS-G156215 | Unicor Federal Prison Industries PVM220PS-IM156215 | Unicor Federal Prison Industries PVM220PS-M156215 | Unicor Federal Prison Industries PVM220PS-Q6LTT215 | Unicor Federal Prison Industries PVM220PS-A2P1220 | Unicor Federal Prison Industries PVM220PS-G156220 | Unicor Federal Prison Industries PVM220PS-IM156220 | Unicor Federal Prison Industries PVM220PS-M156220 | Unicor Federal Prison Industries PVM220PS-Q6LTT220 | Unicor Federal Prison Industries PVM220PS-IM156225 | Unicor Federal Prison Industries PVM220PS-M156225 | Unicor Federal Prison Industries PVM220PS-IM156230 | Unicor Federal Prison Industries PVM220PS-M156230 | Unicor Federal Prison Industries PVM220PS-IM156235 | Unicor Federal Prison Industries PVM220PS-M156235 | Unicor Federal Prison Industries PVM220PS-IM156240 | Universal Energy Nanjing Solar Technology UE M180HR | Universal Energy Nanjing Solar Technology UE M185HR | Universal Energy Nanjing Solar Technology UE M190HR | Universal Energy Nanjing Solar Technology UE P220 | Universal Energy Nanjing Solar Technology UE P225 | Universal Energy Nanjing Solar Technology UE P230 | Universal Energy Nanjing Solar Technology UE P235 | Universal Energy Nanjing Solar Technology UE P240 | Universal Hardware UHC-230M6-6100 | Universal Hardware UHC-230P6-6100 | Universal Hardware UHC-240M6-6100 | Universal Hardware UHC-240P6-6100 | Universal Hardware UHC-250M6-6100 | Universal Hardware UHC-250P6-6100 | Upsolar UP-M155M | Upsolar UP-M160M | Upsolar UP-M165M | Upsolar UP-M170M | Upsolar UP-M175M | Upsolar UP-M175M-B | Upsolar UP-Z175M | Upsolar UP-Z175M-B | Upsolar UP-M180M | Upsolar UP-M180P | Upsolar UP-Z180M | Upsolar UP-Z180M-B | Upsolar UP-M185M | Upsolar UP-M185M-B | Upsolar UP-M185P | Upsolar UP-Z185M | Upsolar UP-Z185M-B | Upsolar UP-M190M | Upsolar UP-M190M-B | Upsolar UP-M190MT | Upsolar UP-M190MT-B | Upsolar UP-M190P | Upsolar UP-S190MT | Upsolar UP-S190MT-B | Upsolar UP-Z190M | Upsolar UP-Z190M-B | Upsolar UP-M195M | Upsolar UP-M195M-B | Upsolar UP-M195P | Upsolar UP-Z195M | Upsolar UP-Z195M-B | Upsolar UP-M200P | Upsolar UP-M205P | Upsolar UP-M205P-B | Upsolar UP-M210P | Upsolar UP-M210P-B | Upsolar UP-M210PT | Upsolar UP-M210PT-B | Upsolar UP-M215P | Upsolar UP-M215P-B | Upsolar UP-M220P | Upsolar UP-M220P-B | Upsolar UP-Z220P | Upsolar UP-Z220P-B | Upsolar UP-M225P | Upsolar UP-Z225P | Upsolar UP-Z225P-B | Upsolar UP-M230M | Upsolar UP-M230M-B | Upsolar UP-M230MS | Upsolar UP-M230MS-B | Upsolar UP-M230MT | Upsolar UP-M230MT-B | Upsolar UP-M230P | Upsolar UP-M230P-B | Upsolar UP-M230PS | Upsolar UP-M230PS-B | Upsolar UP-M230PT | Upsolar UP-M230PT-B | Upsolar UP-Z230M | Upsolar UP-Z230M-B | Upsolar UP-Z230MS | Upsolar UP-Z230MS-B | Upsolar UP-Z230MT | Upsolar UP-Z230MT-B | Upsolar UP-Z230P | Upsolar UP-Z230P-B | Upsolar UP-Z230PS | Upsolar UP-Z230PS-B | Upsolar UP-Z230PT | Upsolar UP-Z230PT-B | Upsolar UP-M235M | Upsolar UP-M235M-B | Upsolar UP-M235MS | Upsolar UP-M235MS-B | Upsolar UP-M235MT | Upsolar UP-M235MT-B | Upsolar UP-M235P | Upsolar UP-M235P-B | Upsolar UP-M235PS | Upsolar UP-M235PS-B | Upsolar UP-M235PT | Upsolar UP-M235PT-B | Upsolar UP-Z235M | Upsolar UP-Z235M-B | Upsolar UP-Z235MS | Upsolar UP-Z235MS-B | Upsolar UP-Z235MT | Upsolar UP-Z235MT-B | Upsolar UP-Z235P | Upsolar UP-Z235P-B | Upsolar UP-Z235PS | Upsolar UP-Z235PS-B | Upsolar UP-Z235PT | Upsolar UP-Z235PT-B | Upsolar UP-M240M | Upsolar UP-M240M-B | Upsolar UP-M240MS | Upsolar UP-M240MS-B | Upsolar UP-M240MT | Upsolar UP-M240MT-B | Upsolar UP-M240P | Upsolar UP-M240P-B | Upsolar UP-M240PS | Upsolar UP-M240PS-B | Upsolar UP-M240PT | Upsolar UP-M240PT-B | Upsolar UP-Z240M | Upsolar UP-Z240M-B | Upsolar UP-Z240MS | Upsolar UP-Z240MS-B | Upsolar UP-Z240MT | Upsolar UP-Z240MT-B | Upsolar UP-Z240P | Upsolar UP-Z240P-B | Upsolar UP-Z240PS | Upsolar UP-Z240PS-B | Upsolar UP-Z240PT | Upsolar UP-Z240PT-B | Upsolar UP-M245M | Upsolar UP-M245M-B | Upsolar UP-M245MS | Upsolar UP-M245MS-B | Upsolar UP-M245MT | Upsolar UP-M245MT-B | Upsolar UP-M245P | Upsolar UP-M245P-B | Upsolar UP-M245PS | Upsolar UP-M245PS-B | Upsolar UP-M245PT | Upsolar UP-M245PT-B | Upsolar UP-Z245M | Upsolar UP-Z245M-B | Upsolar UP-Z245MS | Upsolar UP-Z245MS-B | Upsolar UP-Z245MT | Upsolar UP-Z245MT-B | Upsolar UP-Z245P | Upsolar UP-Z245P-B | Upsolar UP-Z245PS | Upsolar UP-Z245PS-B | Upsolar UP-Z245PT | Upsolar UP-Z245PT-B | Upsolar UP-M250M | Upsolar UP-M250M-B | Upsolar UP-M250MS | Upsolar UP-M250MS-B | Upsolar UP-M250MT | Upsolar UP-M250MT-B | Upsolar UP-M250P | Upsolar UP-M250P-B | Upsolar UP-M250PS | Upsolar UP-M250PS-B | Upsolar UP-M250PT | Upsolar UP-M250PT-B | Upsolar UP-Z250M | Upsolar UP-Z250M-B | Upsolar UP-Z250MS | Upsolar UP-Z250MS-B | Upsolar UP-Z250MT | Upsolar UP-Z250MT-B | Upsolar UP-Z250P | Upsolar UP-Z250P-B | Upsolar UP-Z250PS | Upsolar UP-Z250PS-B | Upsolar UP-Z250PT | Upsolar UP-Z250PT-B | Upsolar UP-M270P | Upsolar UP-M270P-B | Upsolar UP-Z270P | Upsolar UP-Z270P-B | Upsolar UP-M275P | Upsolar UP-M275P-B | Upsolar UP-Z275P | Upsolar UP-Z275P-B | Upsolar UP-M280P | Upsolar UP-M280P-B | Upsolar UP-M280PS | Upsolar UP-M280PT | Upsolar UP-M280PT-B | Upsolar UP-Z280P | Upsolar UP-Z280P-B | Upsolar UP-M285P | Upsolar UP-M285PS | Upsolar UP-M285PT | Upsolar UP-Z285P | Upsolar UP-M290P | Upsolar UP-M290PS | Upsolar UP-M290PT | Upsolar UP-Z290P | Upsolar UP-M295P | Upsolar UP-M295PS | Upsolar UP-M295PT | Upsolar UP-Z295P | Upsolar UP-M300P | Upsolar UP-M300PS | Upsolar UP-M300PT | Upsolar UP-Z300P | US Topco Energy TOPCO-170S5 | US Topco Energy TOPCO-180P6 | US Topco Energy TOPCO-180S5 | US Topco Energy TOPCO-190P6 | US Topco Energy TOPCO-195P6 | US Topco Energy TOPCO-200P6 | US Topco Energy TOPCO-205P6 | US Topco Energy TOPCO-210P6 | US Topco Energy TOPCO-215P6 | US Topco Energy TOPCO-220P6 | US Topco Energy TOPCO-225P6 | US Topco Energy TOPCO-230P6 | US Topco Energy TOPCO-235P6 | US Topco Energy TOPCO-240P6 | US Topco Energy TOPCO-245P6 | US Topco Energy TOPCO-250P6 | US Topco Energy TOPCO-255P6 | US Topco Energy TOPCO-260P6 | US Topco Energy TOPCO-265P6 | US Topco Energy TOPCO-270P6 | US Topco Energy TOPCO-275P6 | US Topco Energy TOPCO-280P6 | US Topco Energy TOPCO-285P6 | Vikram Solar ELDORA 270 | Waaree Energies WU-120 | Waaree Energies WU-125 | Waaree Energies WU-130 | Waaree Energies WSM-135 | Waaree Energies WSM-140 | Waaree Energies WU-140 | Waaree Energies WSM-145 | Waaree Energies WU-175 | Waaree Energies WU-180 | Waaree Energies WU-190 | Waaree Energies WU-200 | Waaree Energies WU-210 | Waaree Energies WS-220 | Waaree Energies WU-220 | Waaree Energies WS-225 | Waaree Energies WS-230 | Waaree Energies WU-230 | Waaree Energies WS-235 | Waaree Energies WS-240 | Waaree Energies WU-240 | Waaree Energies WS-255 | Waaree Energies WS-260 | Waaree Energies WS-265 | Waaree Energies WS-270 | Waaree Energies WS-275 | Waaree Energies WSM-275 | Waaree Energies WS-280 | Waaree Energies WSM-280 | Waaree Energies WS-285 | Waaree Energies WSM-285 | Waaree Energies WS-290 | Waaree Energies WSM-290 | Waaree Energies WSM-295 | Waaree Energies WSM-300 | Waaree Energies WSM-305 | Waaree Energies WSM-310 | Waaree Energies WSM-315 | Wanxiang New Energy WXS175S-US | Wanxiang New Energy WXS180P-US | Wanxiang New Energy WXS180S-US | Wanxiang New Energy WXS185P-US | Wanxiang New Energy WXS185S-US | Wanxiang New Energy WXS190P-US | Wanxiang New Energy WXS200P-US | Wanxiang New Energy WXS205P-US | Wanxiang New Energy WXS210P-US | Wanxiang New Energy WXS215P-US | Wanxiang New Energy WXS220P-US | Wanxiang New Energy WXS225P-US | Wanxiang New Energy WXS230P-US | Wanxiang New Energy WXS235P-US | Wanxiang New Energy WXS240P-US | Wanxiang New Energy WXS245P-US | Wanxiang New Energy WXS250P-US | Wanxiang New Energy WXS255P-US | Wanxiang New Energy WXS260P-US | Wanxiang New Energy WXS265P-US | Wanxiang New Energy WXS270P-US | Wanxiang New Energy WXS275P-US | Wanxiang New Energy WXS280P-US | Wanxiang New Energy WXS285P-US | Watton Solar WTM160M | Watton Solar WTM165M | Watton Solar WTM170M | Watton Solar WTM175M | Watton Solar WTM180M | Watton Solar WTM185M | Watton Solar WTM200P | Watton Solar WTM205P | Watton Solar WTM210P | Watton Solar WTM215P | Watton Solar WTM220P | Watton Solar WTM225P | Watton Solar WTM230P | Watton Solar WTM235P | Watton Solar WTM240P | Webel SL Energy Systems W 1750-170 Wp | Webel SL Energy Systems W 1750-175 Wp | Webel SL Energy Systems W 1750-180 Wp | Webel SL Energy Systems W 2100-210 Wp | Webel SL Energy Systems W 2100-215 Wp | Webel SL Energy Systems W 2100-220 Wp | Webel SL Energy Systems W 2300-230 | Webel SL Energy Systems W 2300-235 Wp | Webel SL Energy Systems W 2300-240 Wp | Websol Energy Systems W2500-250 | Websol Energy Systems W2800-275 | Websol Energy Systems W2800-280 | Websol Energy Systems W2800-285 | Wenzhou Jingri Photovoltaic Technology JRM160M | Wenzhou Jingri Photovoltaic Technology JRM165M | Wenzhou Jingri Photovoltaic Technology JRM170M | Wenzhou Jingri Photovoltaic Technology JRM175M | Wenzhou Jingri Photovoltaic Technology JRM180M | Wenzhou Jingri Photovoltaic Technology JRM185M | Wenzhou Jingri Photovoltaic Technology JRM200P | Wenzhou Jingri Photovoltaic Technology JRM205P | Wenzhou Jingri Photovoltaic Technology JRM210P | Wenzhou Jingri Photovoltaic Technology JRM215P | Wenzhou Jingri Photovoltaic Technology JRM220P | Wenzhou Jingri Photovoltaic Technology JRM225P | Wenzhou Jingri Photovoltaic Technology JRM230P | Wenzhou Jingri Photovoltaic Technology JRM235P | Wenzhou Jingri Photovoltaic Technology JRM240P | Westinghouse Solar ST-165-1 | Westinghouse Solar WS_165_1_DC0_0_B | Westinghouse Solar WS-165-1-DC0-0-A | Westinghouse Solar ST-170-1 | Westinghouse Solar WS_170_1_DC0_0_B | Westinghouse Solar WS-170-1-DC0-0-A | Westinghouse Solar ST-175-1 | Westinghouse Solar WS_175_1_DC0_0_B | Westinghouse Solar WS-175-1AC1-A-A | Westinghouse Solar WS-175-1AC3-B-A | Westinghouse Solar WS-175-1-DC0-0-A | Westinghouse Solar ST-180-1 | Westinghouse Solar WS_180_1_DC0_0_B | Westinghouse Solar WS-180-1-DC0-0-A | Westinghouse Solar ST-185-1 | Westinghouse Solar WS_185_1_DC0_0_A | Westinghouse Solar WS_185_1_DC0_0_B | Westinghouse Solar WS-185-1AC1-A-A | Westinghouse Solar WS-185-1AC1-A-B | Westinghouse Solar WS-185-1AC3-B-A | Westinghouse Solar WS-185-1AC3-B-B | Westinghouse Solar WS_190_1_DC0_0_B | Westinghouse Solar WS-190-1AC1-A-B | Westinghouse Solar WS-190-1AC3-B-B | Westinghouse Solar WS_195_1_DC0_0_B | Westinghouse Solar WS-195-1AC1-A-B | Westinghouse Solar WS-195-1AC3-B-B | Westinghouse Solar WLW-230-1-AC0-D-B | Westinghouse Solar WLW-230-1-AC1-A-B | Westinghouse Solar WLW-230-1-AC2-D-B | Westinghouse Solar WLW-230-1-AC3-B-B | Westinghouse Solar WLW-230-1-DC0-0-B | Westinghouse Solar WLW-230-1-DC0-0-BL | Westinghouse Solar WLW-230-1-DC1-0-B | Westinghouse Solar WLW-235-1-AC0-D-B | Westinghouse Solar WLW-235-1-AC1-A-B | Westinghouse Solar WLW-235-1-AC2-D-B | Westinghouse Solar WLW-235-1-AC3-B-B | Westinghouse Solar WLW-235-1-DC0-0-B | Westinghouse Solar WLW-235-1-DC0-0-BL | Westinghouse Solar WLW-235-1-DC1-0-B | Westinghouse Solar WLW-240-1-AC0-D-B | Westinghouse Solar WLW-240-1-AC1-A-B | Westinghouse Solar WLW-240-1-AC2-D-B | Westinghouse Solar WLW-240-1-AC3-B-B | Westinghouse Solar WLW-240-1-DC0-0-B | Westinghouse Solar WLW-240-1-DC0-0-BL | Westinghouse Solar WLW-240-1-DC1-0-B | Westinghouse Solar WTW-240-1-AC2-D-B | Westinghouse Solar WTW-240-1-DC4-0-B | Westinghouse Solar WTW-245-1-AC2-D-B | Westinghouse Solar WTW-245-1-DC4-0-B | Westinghouse Solar WTW-250-1-AC2-D-B | Westinghouse Solar WTW-250-1-DC4-0-B | Westinghouse Solar WS_260_1_DC0_0_B | Westinghouse Solar WS_270_1_DC0_0_B | Westinghouse Solar WS_280_1_DC0_0_B | Westinghouse Solar WS_290_1_DC0_0_B | WINAICO WSP-225P6 | WINAICO WSP-230P6 | WINAICO WSP-235P6 | WINAICO WSP-240P6 | WINAICO WSP-245P6 | WINAICO WSP-250P6 | WINAICO WSP-255P6 | WINAICO WSP-260M6 | WINAICO WSP-260P6 | WINAICO WSP-265M6 | WINAICO WSP-270M6 | WINAICO WSP-275M6 | WINAICO WSP-280M6 | Wuxi Shangpin Solar Energy Science & Technology SPSM-165D | Wuxi Shangpin Solar Energy Science & Technology SPSM-170D | Wuxi Shangpin Solar Energy Science & Technology SPSM-175D | Wuxi Shangpin Solar Energy Science & Technology SPSM-180D | Wuxi Shangpin Solar Energy Science & Technology SPSM-250P | Wuxi Shangpin Solar Energy Science & Technology SPSM-260P | Wuxi Shangpin Solar Energy Science & Technology SPSM-270P | Xian Huanghe Photovoltaic Technology HH180(36)M | Xian Huanghe Photovoltaic Technology HH185(36)M | Xian Huanghe Photovoltaic Technology HH225(30)P | Xian Huanghe Photovoltaic Technology HH230(30)P | Xian Huanghe Photovoltaic Technology HH235(30)P | Xian Huanghe Photovoltaic Technology HH275(36)P | Xian Huanghe Photovoltaic Technology HH280(36)P | Xian Huanghe Photovoltaic Technology HH285(36)P | XL Telecom & Energy XL 30225 | Xunlight XR12-88 | Xunlight XRS18-146 | Xunlight XRS18-150 | Xunlight XRS18-158 | Xunlight XR 36-264 | Xunlight XR36-291 | Xunlight XR36-300 | Xunlight XR38-307 | Xunlight XR36-315 | Xunlight XRU10-71 | Xunlight XRU10-74 | Yingli Energy (China) YL170P-23b | Yingli Energy (China) YL175P-23b | Yingli Energy (China) YL180P-23b | Yingli Energy (China) YL185P-23b | Yingli Energy (China) YL195P-26b | Yingli Energy (China) YL200P-26b | Yingli Energy (China) YL205P-26b | Yingli Energy (China) YL210P-26b | Yingli Energy (China) YL220P-29b | Yingli Energy (China) YL225P-29b | Yingli Energy (China) YL230P-29b | Yingli Energy (China) YL235P-29b | Yingli Energy (China) YL240P-29b | Yingli Energy (China) YL240P-32b | Yingli Energy (China) YL245P-29b | Yingli Energy (China) YL245P-32b | Yingli Energy (China) YL250C-30b | Yingli Energy (China) YL250P-29b | Yingli Energy (China) YL250P-32b | Yingli Energy (China) YL255C-30b | Yingli Energy (China) YL255P-29b | Yingli Energy (China) YL255P-32b | Yingli Energy (China) YL260C-30b | Yingli Energy (China) YL260P-35b | Yingli Energy (China) YL265C-30b | Yingli Energy (China) YL265P-35b | Yingli Energy (China) YL270C-30b | Yingli Energy (China) YL270P-35b | Yingli Energy (China) YL275P-35b | Yingli Energy (China) YL280P-35b | Yingli Energy (China) YL285P-35b | Yingli Energy (China) YL290P-35b | Yingli Energy (China) YL295P-35b | Yingli Energy (China) YL300P-35b | Yingli Energy (China) YL305P-35b | YOCASOL PCA200-C04 | YOCASOL PCB200-C21 | YOCASOL PCA205-C04 | YOCASOL PCB205-C21 | YOCASOL PCA210-C04 | YOCASOL PCB210-C21 | Yunnan Tianda Photovoltaic TD160M5 | Yunnan Tianda Photovoltaic TD165M5 | Yunnan Tianda Photovoltaic TD170M5 | Yunnan Tianda Photovoltaic TD175M5 | Yunnan Tianda Photovoltaic TD180M5 | Zerquest Solar Zp170 | Zhangjiagang City SEG PV SEGM5-72 170W | Zhangjiagang City SEG PV SEGM5-72 175W | Zhangjiagang City SEG PV SEGM5-72 180W | Zhangjiagang City SEG PV SEGM5-72 185W | Zhangjiagang City SEG PV SEGM5-72 190W | Zhangjiagang City SEG PV SEGM6-54 190W | Zhangjiagang City SEG PV SEGM5-72 195W | Zhangjiagang City SEG PV SEGM6-54 195W | Zhangjiagang City SEG PV SEGM6-54 200W | Zhangjiagang City SEG PV SEGM6-60 200W | Zhangjiagang City SEG PV SEGM6-54 205W | Zhangjiagang City SEG PV SEGM6-60 205W | Zhangjiagang City SEG PV SEGM6-54 210W | Zhangjiagang City SEG PV SEGM6-60 210W | Zhangjiagang City SEG PV SEGM6-60 215W | Zhangjiagang City SEG PV SEGM6-60 220W | Zhangjiagang City SEG PV SEGM6-60 225W | Zhangjiagang City SEG PV SEGM5-96 230W | Zhangjiagang City SEG PV SEGM6-60 230W | Zhangjiagang City SEG PV SEGM5-96 235W | Zhangjiagang City SEG PV SEGM6-60 235W | Zhangjiagang City SEG PV SEGM5-96 240W | Zhangjiagang City SEG PV SEGM6-60 240W | Zhangjiagang City SEG PV SEGM5-96 245W | Zhangjiagang City SEG PV SEGM5-96 250W | Zhangjiagang City SEG PV SEGM5-96 255W | Zhangjiagang City SEG PV SEGM6-72 255W | Zhangjiagang City SEG PV SEGP6-72 255W | Zhangjiagang City SEG PV SEGM6-72 260W | Zhangjiagang City SEG PV SEGP6-72 260W | Zhangjiagang City SEG PV SEGM6-72 265W | Zhangjiagang City SEG PV SEGP6-72 265W | Zhangjiagang City SEG PV SEGM6-72 270W | Zhangjiagang City SEG PV SEGP6-72 270W | Zhangjiagang City SEG PV SEGM6-72 275W | Zhangjiagang City SEG PV SEGP6-72 275W | Zhangjiagang City SEG PV SEGM6-72 280W | Zhangjiagang City SEG PV SEGP6-72 280W | Zhangjiagang City SEG PV SEGM6-72 285W | Zhangjiagang City SEG PV SEGP6-72 285W | Zhangjiagang City SEG PV SEGM6-72 290W | Zhangjiagang City SEG PV SEGP6-72 290W | Zhangjiagang City SEG PV SEGM6-72 295W | Zhangjiagang City SEG PV SEGP6-72 295W | Zhangjiagang City SEG PV SEGM6-72 300W | Zhangjiagang City SEG PV SEGP6-72 300W | Zhangjiagang City Sunlink PV SEGP6-54-195 | Zhangjiagang City Sunlink PV SEGP6-54-200 | Zhangjiagang City Sunlink PV SEGP6-54-205 | Zhangjiagang City Sunlink PV SEGP6-60-220 | Zhangjiagang City Sunlink PV SEGP6-60-225 | Zhangjiagang City Sunlink PV SEGP6-60-230 | Zhejiang ERA Solar Technology ESPSA-170 | Zhejiang ERA Solar Technology ESPSA-175 | Zhejiang ERA Solar Technology ESPSA-180 | Zhejiang Global Photovoltaic Technology GSM-155 | Zhejiang Global Photovoltaic Technology GSM-160 | Zhejiang Global Photovoltaic Technology GSM-165 | Zhejiang Global Photovoltaic Technology GSM-170 | Zhejiang Global Photovoltaic Technology GSM-175 | Zhejiang Global Photovoltaic Technology GSM-180 | Zhejiang Global Photovoltaic Technology GSP-230 | Zhejiang Global Photovoltaic Technology GSM-235 | Zhejiang Global Photovoltaic Technology GSP-235 | Zhejiang Global Photovoltaic Technology GSM-240 | Zhejiang Global Photovoltaic Technology GSP-240 | Zhejiang Global Photovoltaic Technology GSM-245 | Zhejiang Global Photovoltaic Technology GSM-250 | Zhejiang Global Photovoltaic Technology GSP-265 | Zhejiang Global Photovoltaic Technology GSP-270 | Zhejiang Global Photovoltaic Technology GSM-275 | Zhejiang Global Photovoltaic Technology GSP-275 | Zhejiang Global Photovoltaic Technology GSM-280 | Zhejiang Global Photovoltaic Technology GSP-280 | Zhejiang Global Photovoltaic Technology GSM-285 | Zhejiang Global Photovoltaic Technology GSP-285 | Zhejiang Global Photovoltaic Technology GSM-290 | Zhejiang Global Photovoltaic Technology GSM-295 | Zhejiang Global Photovoltaic Technology GSM-300 | Zhejiang Global Photovoltaic Technology GSM-305 | Zhejiang Guangyi Optical Energy Technology GYP-150M | Zhejiang Guangyi Optical Energy Technology GYP-170P | Zhejiang Guangyi Optical Energy Technology GYP-175P | Zhejiang Guangyi Optical Energy Technology GYP-180M | Zhejiang Guangyi Optical Energy Technology GYP-180P | Zhejiang Guangyi Optical Energy Technology GYP-185M | Zhejiang Guangyi Optical Energy Technology GYP-185P | Zhejiang Guangyi Optical Energy Technology GYP-190P | Zhejiang Guangyi Optical Energy Technology GYP-200P | Zhejiang Guangyi Optical Energy Technology GYP-210P | Zhejiang Guangyi Optical Energy Technology GYP-220P | Zhejiang Guangyi Optical Energy Technology GYP-225P | Zhejiang Guangyi Optical Energy Technology GYP-230M | Zhejiang Guangyi Optical Energy Technology GYP-230P | Zhejiang Guangyi Optical Energy Technology GYP-235M | Zhejiang Guangyi Optical Energy Technology GYP-240M | Zhejiang Guangyi Optical Energy Technology GYP-245M | Zhejiang Guangyi Optical Energy Technology GYP-250M | Zhejiang Guangyi Optical Energy Technology GYP-265P | Zhejiang Guangyi Optical Energy Technology GYP-270M | Zhejiang Guangyi Optical Energy Technology GYP-270P | Zhejiang Guangyi Optical Energy Technology GYP-280M | Zhejiang Guangyi Optical Energy Technology GYP-280P | Zhejiang Guangyi Optical Energy Technology GYP-285P | Zhejiang Guangyi Optical Energy Technology GYP-290M | Zhejiang Jiutai New Energy JTM175-72M | Zhejiang Jiutai New Energy JTM180-72M | Zhejiang Jiutai New Energy JTM185-72M | Zhejiang Jiutai New Energy JTM200-60P | Zhejiang Jiutai New Energy JTM205-60P | Zhejiang Jiutai New Energy JTM210-60P | Zhejiang Jiutai New Energy JTM215-60P | Zhejiang Jiutai New Energy JTM220-60P | Zhejiang Jiutai New Energy JTM225-60P | Zhejiang Jiutai New Energy JTM230-60P | Zhejiang Jiutai New Energy JTM235-60P | Zhejiang Jiutai New Energy JTM240-60P | Zhejiang Jiutai New Energy JTM270-72P | Zhejiang Jiutai New Energy JTM275-72P | Zhejiang Jiutai New Energy JTM280-72P | Zhejiang Jiutai New Energy JTM285-72P | Zhejiang Kingdom Solar Energy Technic KD-M160 | Zhejiang Kingdom Solar Energy Technic KD-M165 | Zhejiang Kingdom Solar Energy Technic KD-M170 | Zhejiang Kingdom Solar Energy Technic KD-M175 | Zhejiang Kingdom Solar Energy Technic KD-M180 | Zhejiang Kingdom Solar Energy Technic KD-M185 | Zhejiang Kingdom Solar Energy Technic KD-M190 | Zhejiang Kingdom Solar Energy Technic KD-M195 | Zhejiang Kingdom Solar Energy Technic KD-M200 | Zhejiang Kingdom Solar Energy Technic KD-P200 | Zhejiang Kingdom Solar Energy Technic KD-P205 | Zhejiang Kingdom Solar Energy Technic KD-P210 | Zhejiang Kingdom Solar Energy Technic KD-P215 | Zhejiang Kingdom Solar Energy Technic KD-P220 | Zhejiang Kingdom Solar Energy Technic KD-P225 | Zhejiang Kingdom Solar Energy Technic KD-P230 | Zhejiang Kingdom Solar Energy Technic KD-P235 | Zhejiang Kingdom Solar Energy Technic KD-P240 | Zhejiang Kingdom Solar Energy Technic KD-P245 | Zhejiang Kingdom Solar Energy Technic KD-P250 | Zhejiang Kingdom Solar Energy Technic KD-P255 | Zhejiang Kingdom Solar Energy Technic KD-P260 | Zhejiang Kingdom Solar Energy Technic KD-P265 | Zhejiang Kingdom Solar Energy Technic KD-P270 | Zhejiang Kingdom Solar Energy Technic KD-P275 | Zhejiang Kingdom Solar Energy Technic KD-P280 | Zhejiang Kingdom Solar Energy Technic KD-P285 | Zhejiang Kingdom Solar Energy Technic KD-P290 | Zhejiang Kingdom Solar Energy Technic KD-P295 | Zhejiang Kingdom Solar Energy Technic KD-P300 | Zhejiang Shinew Photoelectronic Technology XH-72M-185 | Zhejiang Shinew Photoelectronic Technology XH-72M-190 | Zhejiang Shinew Photoelectronic Technology XH-60P-230 | Zhejiang Shinew Photoelectronic Technology XH-60P-235 | Zhejiang Shinew Photoelectronic Technology XH-72P-280 | ZheJiang SOCO Technology SC180M-24-P | ZheJiang SOCO Technology SC230M-24-J | ZheJiang SOCO Technology SC230P-24-B | ZheJiang SOCO Technology SC275P-24-A | ZheJiang SOCO Technology SC280M-24-H | Zhejiang Sunflower Light Energy Science & Tech SF125x125-72-M-150W | Zhejiang Sunflower Light Energy Science & Tech SF125x125-72-M-155W | Zhejiang Sunflower Light Energy Science & Tech SF125x125-72-M-160W | Zhejiang Sunflower Light Energy Science & Tech SF125x125-72-M-165W | Zhejiang Sunflower Light Energy Science & Tech SF125x125-72-M-170W | Zhejiang Sunflower Light Energy Science & Tech SF125x125-72-M-175W | Zhejiang Sunflower Light Energy Science & Tech SF125x125-72-M-180W | Zhejiang Sunflower Light Energy Science & Tech SF125x125-72-M-185W | Zhejiang Sunflower Light Energy Science & Tech SF156x156-60-M-200W | Zhejiang Sunflower Light Energy Science & Tech SF156x156-60-P-200W | Zhejiang Sunflower Light Energy Science & Tech SF156x156-60-M-205W | Zhejiang Sunflower Light Energy Science & Tech SF156x156-60-P-205W | Zhejiang Sunflower Light Energy Science & Tech SF156x156-60-M-210W | Zhejiang Sunflower Light Energy Science & Tech SF156x156-60-P-210W | Zhejiang Sunflower Light Energy Science & Tech SF156x156-60-M-215W | Zhejiang Sunflower Light Energy Science & Tech SF156x156-60-P-215W | Zhejiang Sunflower Light Energy Science & Tech SF156x156-60-M-220W | Zhejiang Sunflower Light Energy Science & Tech SF156x156-60-P-220W | Zhejiang Sunflower Light Energy Science & Tech SF156x156-60-M-225W | Zhejiang Sunflower Light Energy Science & Tech SF156x156-60-P-225W | Zhejiang Sunflower Light Energy Science & Tech SF156x156-60-M-230W | Zhejiang Sunflower Light Energy Science & Tech SF156x156-60-P-230W | Zhejiang Sunflower Light Energy Science & Tech SF156x156-60-M-235W | Zhejiang Sunflower Light Energy Science & Tech SF156x156-60-M-240W | Zhejiang Wanxiang Solar WXS175P | Zhejiang Wanxiang Solar WXS175S | Zhejiang Wanxiang Solar WXS180P | Zhejiang Wanxiang Solar WXS180S | Zhejiang Wanxiang Solar WXS185P | Zhejiang Wanxiang Solar WXS185S | Zhejiang Wanxiang Solar WXS190P | Zhejiang Wanxiang Solar WXS200P | Zhejiang Wanxiang Solar WXS205P | Zhejiang Wanxiang Solar WXS210P | Zhejiang Wanxiang Solar WXS215P | Zhejiang Wanxiang Solar WXS220P | Zhejiang Wanxiang Solar WXS225P | Zhejiang Wanxiang Solar WXS230P | Zhejiang Wanxiang Solar WXS235P | Zhejiang Wanxiang Solar WXS240P | Zhejiang Wanxiang Solar WXS245P | Zhejiang Wanxiang Solar WXS250P | Zhejiang Wanxiang Solar WXS255P | Zhejiang Wanxiang Solar WXS260P | Zhejiang Wanxiang Solar WXS265P | Zhejiang Wanxiang Solar WXS270P | Zhejiang Wanxiang Solar WXS275P | Zhejiang Wanxiang Solar WXS280P | Zhongli Talesun Solar TP572M-175 | Zhongli Talesun Solar TP572M-180 | Zhongli Talesun Solar TP572M-185 | Zhongli Talesun Solar TP572M-190 | Zhongli Talesun Solar TP572M-195 | Zhongli Talesun Solar TP572M-200 | Zhongli Talesun Solar TP660M-220 | Zhongli Talesun Solar TP660P-220 | Zhongli Talesun Solar TP660M-225 | Zhongli Talesun Solar TP660P-225 | Zhongli Talesun Solar TP660M-230 | Zhongli Talesun Solar TP660P-230 | Zhongli Talesun Solar TP660M-235 | Zhongli Talesun Solar TP660P-235 | Zhongli Talesun Solar TP660M-240 | Zhongli Talesun Solar TP660P-240 | Zhongli Talesun Solar TP660M-245 | Zhongli Talesun Solar TP660P-245 | Zhongli Talesun Solar TAC208-240 | Zhongli Talesun Solar TP660M-250 | Zhongli Talesun Solar TP660P-250 | Zhongli Talesun Solar TP660M-255 | Zhongli Talesun Solar TP660P-255 | Zhongli Talesun Solar TP660M-260 | Zhongli Talesun Solar TP672P-280 | Zhongli Talesun Solar TP672M-285 | Zhongli Talesun Solar TP672P-285 | Zhongli Talesun Solar TP672M-290 | Zhongli Talesun Solar TP672P-290 | Zhongli Talesun Solar TP672M-295 | Zhongli Talesun Solar TP672P-295 | Zhongli Talesun Solar TP672M-300 | Zhongli Talesun Solar TP672P-300 | Zhongli Talesun Solar TP672M-305 | Zhongli Talesun Solar TP672M-310 | Znshine PV-Tech ZX175(36)MS | Znshine PV-Tech ZX180(36)MS | Znshine PV-Tech ZX185(36)MS | Znshine PV-Tech ZX190(36)MS | Znshine PV-Tech ZX195(36)MS | Znshine PV-Tech ZX200(36)MS | Znshine PV-Tech ZXM5-72-205-MS | Znshine PV-Tech ZXM5-72-210-MS | Znshine PV-Tech ZXM5-72-215-MS | Znshine PV-Tech ZX220(30)P | Znshine PV-Tech ZX225(30)P | Znshine PV-Tech ZXM6-60-225-M | Znshine PV-Tech ZX230(30)P | Znshine PV-Tech ZXM6-60-230-M | Znshine PV-Tech ZX235(30)P | Znshine PV-Tech ZXM6-60-235-M | Znshine PV-Tech ZX240(30)P | Znshine PV-Tech ZXM6-60-240-M | Znshine PV-Tech ZX245(30)P | Znshine PV-Tech ZX245(48)MS | Znshine PV-Tech ZXM6-60-245-M | Znshine PV-Tech ZX250(48)MS | Znshine PV-Tech ZXM6-60-250-M | Znshine PV-Tech ZXP6-60-250-P | Znshine PV-Tech ZX255(48)MS | Znshine PV-Tech ZXM6-60-255-M | Znshine PV-Tech ZXP6-60-255-P | Znshine PV-Tech ZX260(48)MS | Znshine PV-Tech ZXM6-60-260-M | Znshine PV-Tech ZXP6-60-260-P | Znshine PV-Tech ZX265(36)P | Znshine PV-Tech ZX265(48)MS | Znshine PV-Tech ZXM6-60-265-M | Znshine PV-Tech ZXM6-72-265-M | Znshine PV-Tech ZX270(36)P | Znshine PV-Tech ZX270(48)MS | Znshine PV-Tech ZXM6-60-270-M | Znshine PV-Tech ZXM6-72-270-M | Znshine PV-Tech ZX275(36)P | Znshine PV-Tech ZX275(48)MS | Znshine PV-Tech ZXM6-72-275-M | Znshine PV-Tech ZX280(36)P | Znshine PV-Tech ZXM5-96-280-MS | Znshine PV-Tech ZXM6-72-280-M | Znshine PV-Tech ZX285(36)P | Znshine PV-Tech ZXM5-96-285-MS | Znshine PV-Tech ZXM6-72-285-M | Znshine PV-Tech ZX290(36)P | Znshine PV-Tech ZXM6-72-290-M | Znshine PV-Tech ZX295(36)P | Znshine PV-Tech ZXM6-72-295-M | Znshine PV-Tech ZXM6-72-300-M | Znshine PV-Tech ZXP6-72-300-P | Znshine PV-Tech ZXM6-72-305-M | Znshine PV-Tech ZXP6-72-305-P | Znshine PV-Tech ZXM6-72-310-M | Znshine PV-Tech ZXP6-72-310-P | Znshine PV-Tech ZXM6-72-315-M | Znshine PV-Tech ZXP6-72-315-P | Znshine PV-Tech ZXM6-72-320-M | Znshine PV-Tech ZXM6-72-325-M | Znshine PV-Tech ZXM6-72-330-M | Zytech Engineering Technology ZT170S | Zytech Engineering Technology ZT175S | Zytech Engineering Technology ZT180S | Zytech Engineering Technology ZT185S | Zytech Engineering Technology ZT190S
      mask Callback ModuleName: PVArrayCback(gcb)
      mask Callback BAL: PVArrayCback(gcb)
      mask DialogControl PlotButton Prompt: Plot
      mask DialogControl PlotButton Callback: PVArrayPlot(gcb,'detailed')
      mask DialogControl Container9 Prompt: Measurement Filter
      mask DialogControl Disabled Prompt: - Disabled
      mask DialogControl EnabledDisc Prompt: - Enabled,  using a time constant of 10*(Powergui sample time)
      mask Display:
      | image(imread('panel.jpg'))
      | color('yellow')
      | port_label('input',1,'Ir')
      | port_label('input',2,'T')
      | port_label('output',1,'m')
      | port_label('output',1,'m')
      | port_label('Rconn',1,'+')
      | port_label('Rconn',2,'-')
  Conn1 : PMIOPort  Port=1  Side=Right
  Conn2 : PMIOPort  Port=2  Side=Right
  Out : Outport
  wires:
  PV Array/1(m) -> Out/1
  "      "/1 -> PV Array/1(S)
  "Irradiance "/1(Ir) -> "      "/2
  Constant/1 -> "      "/1
  "      1"/1 -> PV Array/2(TempC)
  "Irradiance "/2(Temp) -> "      1"/1
  Constant1/1 -> "      1"/2
  connections:
  PV Array/RConn1 -- Conn1/RConn1
  PV Array/RConn2 -- Conn2/RConn1
